simulink model "Finalannfaultdetecandclass"  (R2024b)
settings: Solver=ode45  StartTime=0.0  StopTime=0.4  FixedStep=1e-6  MaxStep=0.04  RelTol=1e-3  EnableMultiTasking=on
PreLoadFcn:
  | power_13NodeTestFeeder_init;
values from neighbouring files (symbols this model uses):
  C_601 = [1.03835973183e-08  -3.28956213337e-09  -2.07596127216e-09; -3.28956213337e-09  9.8230300863e-09  -1.22250137004e-09; -2.07596127216e-09  -1.22250137004e-09  9.29377945947e-09]    [Finalmat.mat]    (also in bus1.mat; bus10.mat; bus11.mat; bus12.mat)
  C_602 = [9.39333329896e-09  -1.78290377777e-09  -2.78635373607e-09; -1.78290377777e-09  8.5370713848e-09  -1.08586207709e-09; -2.78635373607e-09  -1.08586207709e-09  8.94105559107e-09]    [Finalmat.mat]    (also in bus1.mat; bus10.mat; bus11.mat; bus12.mat)
  C_603 = [0  0  0; 0  7.76272711671e-09  -1.48325331387e-09; 0  -1.48325331387e-09  7.69036927641e-09]    [Finalmat.mat]    (also in bus1.mat; bus10.mat; bus11.mat; bus12.mat)
  C_604 = [7.69036927641e-09  0  -1.48325331387e-09; 0  0  0; -1.48325331387e-09  0  7.76272711671e-09]    [Finalmat.mat]    (also in bus1.mat; bus10.mat; bus11.mat; bus12.mat)
  C_605 = [0  0  0; 0  0  0; 0  0  7.44890176838e-09]    [Finalmat.mat]    (also in bus1.mat; bus10.mat; bus11.mat; bus12.mat)
  C_606 = [1.59697709306e-07  -1.64824237567e-15  -1.64824237567e-15; -1.64824237567e-15  1.59697709306e-07  -1.64824237567e-15; -1.64824237567e-15  -1.64824237567e-15  1.59697709306e-07]    [Finalmat.mat]    (also in bus1.mat; bus10.mat; bus11.mat; bus12.mat)
  C_607 = [1.46679066902e-07  0  0; 0  0  0; 0  0  0]    [Finalmat.mat]    (also in bus1.mat; bus10.mat; bus11.mat; bus12.mat)
  ft2km = 0.0003048    [Finalmat.mat]    (also in bus1.mat; bus10.mat; bus11.mat; bus12.mat)
  L_601 = [0.0016777459142  0.000826923199875  0.000698195470335; 0.000826923199875  0.00172702836123  0.000634408490396; 0.000698195470335  0.000634408490396  0.00170560121035]    [Finalmat.mat]    (also in bus1.mat; bus10.mat; bus11.mat; bus12.mat)
  L_602 = [0.00194723354262  0.000698195470335  0.000826923199875; 0.000698195470335  0.00197508883877  0.000634408490396; 0.000826923199875  0.000634408490396  0.00199635116541]    [Finalmat.mat]    (also in bus1.mat; bus10.mat; bus11.mat; bus12.mat)
  L_603 = [0  0  0; 0  0.00222034730427  0.000756708074671; 0  0.000756708074671  0.00223650007955]    [Finalmat.mat]    (also in bus1.mat; bus10.mat; bus11.mat; bus12.mat)
  L_604 = [0.00223650007955  0  0.000756708074671; 0  0  0; 0.000756708074671  0  0.00222034730427]    [Finalmat.mat]    (also in bus1.mat; bus10.mat; bus11.mat; bus12.mat)
  L_605 = [0  0  0; 0  0  0; 0  0  0.00222100660122]    [Finalmat.mat]    (also in bus1.mat; bus10.mat; bus11.mat; bus12.mat)
  L_606 = [0.000735610572263  5.40623499221e-05  2.35698659721e-05; 5.40623499221e-05  0.000666054744009  5.40623499221e-05; 2.35698659721e-05  5.40623499221e-05  0.000735610572263]    [Finalmat.mat]    (also in bus1.mat; bus10.mat; bus11.mat; bus12.mat)
  L_607 = [0.000844559393295  0  0; 0  0  0; 0  0  0]    [Finalmat.mat]    (also in bus1.mat; bus10.mat; bus11.mat; bus12.mat)
  R_601 = [0.215305653249  0.0969341469174  0.0981768923907; 0.0969341469174  0.209713298619  0.0953807150757; 0.0981768923907  0.0953807150757  0.212136652292]    [Finalmat.mat]    (also in bus1.mat; bus10.mat; bus11.mat; bus12.mat)
  R_602 = [0.467645121603  0.0981768923907  0.0969341469174; 0.0981768923907  0.464476120646  0.0953807150757; 0.0969341469174  0.0953807150757  0.462052766973]    [Finalmat.mat]    (also in bus1.mat; bus10.mat; bus11.mat; bus12.mat)
  R_603 = [0  0  0; 0  0.826052916102  0.128375607392; 0  0.128375607392  0.822573228777]    [Finalmat.mat]    (also in bus1.mat; bus10.mat; bus11.mat; bus12.mat)
  R_604 = [0.822573228777  0  0.128375607392; 0  0  0; 0.128375607392  0  0.826052916102]    [Finalmat.mat]    (also in bus1.mat; bus10.mat; bus11.mat; bus12.mat)
  R_605 = [0  0  0; 0  0  0; 0  0  0.825928641555]    [Finalmat.mat]    (also in bus1.mat; bus10.mat; bus11.mat; bus12.mat)
  R_606 = [0.495979718394  0.198342177539  0.177029092672; 0.198342177539  0.49032522649  0.198342177539; 0.177029092672  0.198342177539  0.495979718394]    [Finalmat.mat]    (also in bus1.mat; bus10.mat; bus11.mat; bus12.mat)
  R_607 = [0.834192898952  0  0; 0  0  0; 0  0  0]    [Finalmat.mat]    (also in bus1.mat; bus10.mat; bus11.mat; bus12.mat)
libraries: neural x123, spsLoadFlowBusLib x12, spsDistributedParametersLineLib x9, spsThreePhaseSeriesRLCLoadLib x7, spsMultimeterLib x6, spsPowerPhasorLib x6, spsSeriesRLCLoadLib x5, spsThreePhaseVIMeasurementLib x4, spsGroundLib x4, spsThreePhaseSourceLib x1, spsThreePhaseBreakerLib x1, simulink x1
(part 3 of 4)

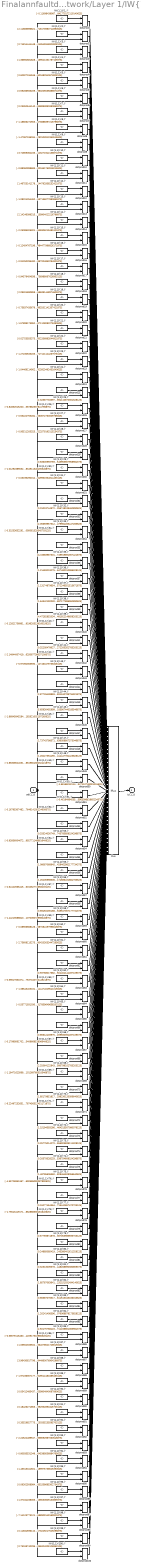
== system Finalannfaultdetecandclass/Subsystem1/Function Fitting Neural Network/Layer 1/IW{1,1} ==
  "pd{1,1}" : Inport  PortDimensions=9
      mask Display: e = 0.06;c1 = [120 230 180]/255;c2 = ([120 230 180]+0)/(256+128);c3 = ([120 230 180]+128)/(256+128);patch([0 1 1 0],[0 0 1 1],c1);patch([0 1 1 1-e 1-e 0+e],[0 0 1 1-e 0+e 0+e],c2);patch([0 0 1 1-e 0+e 0+e],[0 1 1 1-e 1-e 0+e],c3);plot([0 1 1 0 0],[0 0 1 1 0]);
  "IW{1,1}(1,:)'" : Constant  Value=[-0.1169843998710173860189343031379394233226776123046875;-0.315271633824277086599607855532667599618434906005859375;0.79107230882120094239695617943652905523777008056640625;2.164746661655950532576753175817430019378662109375;2.22846879307639600398260881775058805942535400390625;-0.496204760157834379175056938038324005901813507080078125;0.789299834193724958453231010935269296169281005859375;1.6089462914118823899656263165525160729885101318359375;1.6317914608558441447172526750364340841770172119140625]
      mask Display: e = 0.06;c1 = [120 150 230]/255;c2 = ([120 150 230]+0)/383;c3 = ([120 150 230]+128)/383;patch([0 1 1 0],[0 0 1 1],c1);patch([0 1 1 1-e 1-e 0+e],[0 0 1 1-e 0+e 0+e],c2);patch([0 0 1 1-e 0+e 0+e],[0 1 1 1-e 1-e 0+e],c3);plot([0 1 1 0 0],[0 0 1 1 0]);disp('Weights');
  "IW{1,1}(10,:)'" : Constant  Value=[3.7285906223340621323814048082567751407623291015625;-5.223607369509156939102467731572687625885009765625;-3.877261867529044447877595302998088300228118896484375;-2.37152119563655094935938905109651386737823486328125;0.346269172224675625404444190280628390610218048095703125;0.249853727006402959176512013073079288005828857421875;2.016518874910780301235035949503071606159210205078125;0.12714323667959070984778691126848571002483367919921875;3.85153838870149467510373142431490123271942138671875]
      mask Display: e = 0.06;c1 = [120 150 230]/255;c2 = ([120 150 230]+0)/383;c3 = ([120 150 230]+128)/383;patch([0 1 1 0],[0 0 1 1],c1);patch([0 1 1 1-e 1-e 0+e],[0 0 1 1-e 0+e 0+e],c2);patch([0 0 1 1-e 0+e 0+e],[0 1 1 1-e 1-e 0+e],c3);plot([0 1 1 0 0],[0 0 1 1 0]);disp('Weights');
  "IW{1,1}(100,:)'" : Constant  Value=[0.75159740295858845637866352262790314853191375732421875;0.611763010254613437410853293840773403644561767578125;-1.1757815630723575939242664389894343912601470947265625;-0.3695637396224269455302646747441031038761138916015625;-1.00856355672777286969221677281893789768218994140625;-1.17072870773329018589947736472822725772857666015625;-0.284274780055891851393568003913969732820987701416015625;-0.27928563589691524082780915705370716750621795654296875;-0.460633928950748672281889639634755440056324005126953125]
      mask Display: e = 0.06;c1 = [120 150 230]/255;c2 = ([120 150 230]+0)/383;c3 = ([120 150 230]+128)/383;patch([0 1 1 0],[0 0 1 1],c1);patch([0 1 1 1-e 1-e 0+e],[0 0 1 1-e 0+e 0+e],c2);patch([0 0 1 1-e 0+e 0+e],[0 1 1 1-e 1-e 0+e],c3);plot([0 1 1 0 0],[0 0 1 1 0]);disp('Weights');
  "IW{1,1}(11,:)'" : Constant  Value=[-0.8806299868369491523623082684935070574283599853515625;0.30294503373344217056484239947167225182056427001953125;-0.985643459112008457623232970945537090301513671875;-1.042790592220203205187090134131722152233123779296875;0.03439230691604992784515815174017916433513164520263671875;-0.7663674282703316631426559979445300996303558349609375;-0.1309829792505974033200999429027433507144451141357421875;1.19695760712173449036299643921665847301483154296875;-0.603326884093489557159273317665793001651763916015625]
      mask Display: e = 0.06;c1 = [120 150 230]/255;c2 = ([120 150 230]+0)/383;c3 = ([120 150 230]+128)/383;patch([0 1 1 0],[0 0 1 1],c1);patch([0 1 1 1-e 1-e 0+e],[0 0 1 1-e 0+e 0+e],c2);patch([0 0 1 1-e 0+e 0+e],[0 1 1 1-e 1-e 0+e],c3);plot([0 1 1 0 0],[0 0 1 1 0]);disp('Weights');
  "IW{1,1}(12,:)'" : Constant  Value=[1.467531411784743777815265275421552360057830810546875;0.81942273041387891918674313274095766246318817138671875;-0.426906460314266433808683132156147621572017669677734375;0.0749099326592369274546712176743312738835811614990234375;0.2767354436636242365210591742652468383312225341796875;-0.44931784033513844089924305080785416066646575927734375;-1.3652143765277269249480696089449338614940643310546875;-0.9067069902855917629125315215787850320339202880859375;1.80456787422012165933438154752366244792938232421875]
      mask Display: e = 0.06;c1 = [120 150 230]/255;c2 = ([120 150 230]+0)/383;c3 = ([120 150 230]+128)/383;patch([0 1 1 0],[0 0 1 1],c1);patch([0 1 1 1-e 1-e 0+e],[0 0 1 1-e 0+e 0+e],c2);patch([0 0 1 1-e 0+e 0+e],[0 1 1 1-e 1-e 0+e],c3);plot([0 1 1 0 0],[0 0 1 1 0]);disp('Weights');
  "IW{1,1}(13,:)'" : Constant  Value=[-1.0822425445261616427927719996660016477108001708984375;0.1421490865617053567238059486044221557676792144775390625;-0.222184322552897717262254673187271691858768463134765625;-0.808228806975540781110112220630981028079986572265625;-1.0680830130463825344833139752154238522052764892578125;-0.601523564092997897745362934074364602565765380859375;-0.383432119718707775657406955360784195363521575927734375;-0.9219141055654793692752946299151517450809478759765625;0.8695716425988064823826562133035622537136077880859375]
      mask Display: e = 0.06;c1 = [120 150 230]/255;c2 = ([120 150 230]+0)/383;c3 = ([120 150 230]+128)/383;patch([0 1 1 0],[0 0 1 1],c1);patch([0 1 1 1-e 1-e 0+e],[0 0 1 1-e 0+e 0+e],c2);patch([0 0 1 1-e 0+e 0+e],[0 1 1 1-e 1-e 0+e],c3);plot([0 1 1 0 0],[0 0 1 1 0]);disp('Weights');
  "IW{1,1}(14,:)'" : Constant  Value=[2.142460993155533177656479892903007566928863525390625;10.1614423157743711811917819431982934474945068359375;3.70307782718048716930070440866984426975250244140625;-3.40332227325013025875932726194150745868682861328125;-4.92901742923601204893202520906925201416015625;-0.3106434304567471382796384204993955790996551513671875;0.36314955798367598571729786272044293582439422607421875;-1.5022598816808301336322983843274414539337158203125;-0.85323991640809271341794328691321425139904022216796875]
      mask Display: e = 0.06;c1 = [120 150 230]/255;c2 = ([120 150 230]+0)/383;c3 = ([120 150 230]+128)/383;patch([0 1 1 0],[0 0 1 1],c1);patch([0 1 1 1-e 1-e 0+e],[0 0 1 1-e 0+e 0+e],c2);patch([0 0 1 1-e 0+e 0+e],[0 1 1 1-e 1-e 0+e],c3);plot([0 1 1 0 0],[0 0 1 1 0]);disp('Weights');
  "IW{1,1}(15,:)'" : Constant  Value=[-2.250853263014513050421783191268332302570343017578125;-1.5675733809487208958444171003066003322601318359375;-2.639720797748891012446392778656445443630218505859375;-1.129364156634995453032388468272984027862548828125;-0.1049300748916680847688809308237978257238864898681640625;-0.46033186696821670746970767140737734735012054443359375;-0.52897352207262049450520180471357889473438262939453125;-0.6865105178810761987762134594959206879138946533203125;-0.829512207131862577824676918680779635906219482421875]
      mask Display: e = 0.06;c1 = [120 150 230]/255;c2 = ([120 150 230]+0)/383;c3 = ([120 150 230]+128)/383;patch([0 1 1 0],[0 0 1 1],c1);patch([0 1 1 1-e 1-e 0+e],[0 0 1 1-e 0+e 0+e],c2);patch([0 0 1 1-e 0+e 0+e],[0 1 1 1-e 1-e 0+e],c3);plot([0 1 1 0 0],[0 0 1 1 0]);disp('Weights');
  "IW{1,1}(16,:)'" : Constant  Value=[-0.124547671966561968037723318047937937080860137939453125;-0.97962320291865012666931988860596902668476104736328125;-0.77587019687066904882755125072435475885868072509765625;-0.79405829690015672372993549288366921246051788330078125;0.908115781658020981836898499750532209873199462890625;-1.15023286167464533491511247120797634124755859375;-0.72788619861410641664889453750220127403736114501953125;-0.6258857474855545888203778304159641265869140625;-0.86503298797361949379336465426604263484477996826171875]
      mask Display: e = 0.06;c1 = [120 150 230]/255;c2 = ([120 150 230]+0)/383;c3 = ([120 150 230]+128)/383;patch([0 1 1 0],[0 0 1 1],c1);patch([0 1 1 1-e 1-e 0+e],[0 0 1 1-e 0+e 0+e],c2);patch([0 0 1 1-e 0+e 0+e],[0 1 1 1-e 1-e 0+e],c3);plot([0 1 1 0 0],[0 0 1 1 0]);disp('Weights');
  "IW{1,1}(17,:)'" : Constant  Value=[-0.9125029549285799124191953524132259190082550048828125;0.65789174760089685900510403371299616992473602294921875;-0.3630280915494610294302901820628903806209564208984375;-1.5262397482698377704224412809708155691623687744140625;0.382282968203021045194844873549300245940685272216796875;-0.50109375420562629610543581293313764035701751708984375;0.403398421119719186034302538246265612542629241943359375;-1.0463958350801878527391863826778717339038848876953125;0.13938267986139585286053943491424433887004852294921875]
      mask Display: e = 0.06;c1 = [120 150 230]/255;c2 = ([120 150 230]+0)/383;c3 = ([120 150 230]+128)/383;patch([0 1 1 0],[0 0 1 1],c1);patch([0 1 1 1-e 1-e 0+e],[0 0 1 1-e 0+e 0+e],c2);patch([0 0 1 1-e 0+e 0+e],[0 1 1 1-e 1-e 0+e],c3);plot([0 1 1 0 0],[0 0 1 1 0]);disp('Weights');
  "IW{1,1}(18,:)'" : Constant  Value=[-0.94579454836057330613385829565231688320636749267578125;-0.481903233177059575620404530127416364848613739013671875;-1.294686789832062867589002053136937320232391357421875;-1.1112375364712818726076193343033082783222198486328125;0.4852736235741639259089197366847656667232513427734375;-0.31209665885055015710491943536908365786075592041015625;-0.475487892830769587337869097609655000269412994384765625;-0.76513410578662643946046273413230665028095245361328125;0.6284181733856375462465848613646812736988067626953125]
      mask Display: e = 0.06;c1 = [120 150 230]/255;c2 = ([120 150 230]+0)/383;c3 = ([120 150 230]+128)/383;patch([0 1 1 0],[0 0 1 1],c1);patch([0 1 1 1-e 1-e 0+e],[0 0 1 1-e 0+e 0+e],c2);patch([0 0 1 1-e 0+e 0+e],[0 1 1 1-e 1-e 0+e],c3);plot([0 1 1 0 0],[0 0 1 1 0]);disp('Weights');
  "IW{1,1}(19,:)'" : Constant  Value=[2.09324690859917073026963407755829393863677978515625;1.8545893594789186753502008286886848509311676025390625;3.40226567513793387576015447848476469516754150390625;1.990023753797214300931273101014085114002227783203125;3.124260085397577046961714586359448730945587158203125;3.325679193829385926761688097030855715274810791015625;2.143373231000686107705632821307517588138580322265625;4.98029780353131013015399730647914111614227294921875;-0.0279620074952092421971538982461424893699586391448974609375]
      mask Display: e = 0.06;c1 = [120 150 230]/255;c2 = ([120 150 230]+0)/383;c3 = ([120 150 230]+128)/383;patch([0 1 1 0],[0 0 1 1],c1);patch([0 1 1 1-e 1-e 0+e],[0 0 1 1-e 0+e 0+e],c2);patch([0 0 1 1-e 0+e 0+e],[0 1 1 1-e 1-e 0+e],c3);plot([0 1 1 0 0],[0 0 1 1 0]);disp('Weights');
  "IW{1,1}(2,:)'" : Constant  Value=[2.118838968214732165762370641459710896015167236328125;1.8422898698446019682961605212767608463764190673828125;1.7253980455788096026736866406281478703022003173828125;2.312711415512553880802215644507668912410736083984375;1.633846170213174797680721894721500575542449951171875;3.367708596197346526679439193685539066791534423828125;-0.477140207343875910606101342636975459754467010498046875;2.613116127417966172430396909476257860660552978515625;2.66044281460288178919881829642690718173980712890625]
      mask Display: e = 0.06;c1 = [120 150 230]/255;c2 = ([120 150 230]+0)/383;c3 = ([120 150 230]+128)/383;patch([0 1 1 0],[0 0 1 1],c1);patch([0 1 1 1-e 1-e 0+e],[0 0 1 1-e 0+e 0+e],c2);patch([0 0 1 1-e 0+e 0+e],[0 1 1 1-e 1-e 0+e],c3);plot([0 1 1 0 0],[0 0 1 1 0]);disp('Weights');
  "IW{1,1}(20,:)'" : Constant  Value=[-0.75837435679497067209098304374492727220058441162109375;-0.6892949176616320894339651204063557088375091552734375;0.753111799274041260332523961551487445831298828125;-0.91091131319990059633795453919447027146816253662109375;-1.5778653536172468907494703671545721590518951416015625;0.196715916355157671713271838598302565515041351318359375;-0.741954547816795706438597335363738238811492919921875;-0.72451613103801992821217936580069363117218017578125;0.1524088000274099463648980190555448643863201141357421875]
      mask Display: e = 0.06;c1 = [120 150 230]/255;c2 = ([120 150 230]+0)/383;c3 = ([120 150 230]+128)/383;patch([0 1 1 0],[0 0 1 1],c1);patch([0 1 1 1-e 1-e 0+e],[0 0 1 1-e 0+e 0+e],c2);patch([0 0 1 1-e 0+e 0+e],[0 1 1 1-e 1-e 0+e],c3);plot([0 1 1 0 0],[0 0 1 1 0]);disp('Weights');
  "IW{1,1}(21,:)'" : Constant  Value=[-1.5789917395288621815296892236801795661449432373046875;1.214552039187205334513919297023676335811614990234375;3.73117140937676605716433186898939311504364013671875;0.77037511306426853519013775439816527068614959716796875;1.5764585080023330032616968310321681201457977294921875;2.01224664776738659810462195309810340404510498046875;2.796831728956418405829253970296122133731842041015625;1.3456250197286101499827282168553210794925689697265625;-1.00351996366601614596447689109481871128082275390625]
      mask Display: e = 0.06;c1 = [120 150 230]/255;c2 = ([120 150 230]+0)/383;c3 = ([120 150 230]+128)/383;patch([0 1 1 0],[0 0 1 1],c1);patch([0 1 1 1-e 1-e 0+e],[0 0 1 1-e 0+e 0+e],c2);patch([0 0 1 1-e 0+e 0+e],[0 1 1 1-e 1-e 0+e],c3);plot([0 1 1 0 0],[0 0 1 1 0]);disp('Weights');
  "IW{1,1}(22,:)'" : Constant  Value=[0.0275355537349462921314913188552964129485189914703369140625;1.226104677340150050923739399877376854419708251953125;1.3106202217751985461546837541391141712665557861328125;1.232110528501700219550230031018145382404327392578125;-0.31173567352762432403068260100553743541240692138671875;0.09857858649987212562582072905570385046303272247314453125;0.329183085854514778656465523454244248569011688232421875;-0.5875847517893213467488067180966027081012725830078125;-0.6811877548597073950276126197422854602336883544921875]
      mask Display: e = 0.06;c1 = [120 150 230]/255;c2 = ([120 150 230]+0)/383;c3 = ([120 150 230]+128)/383;patch([0 1 1 0],[0 0 1 1],c1);patch([0 1 1 1-e 1-e 0+e],[0 0 1 1-e 0+e 0+e],c2);patch([0 0 1 1-e 0+e 0+e],[0 1 1 1-e 1-e 0+e],c3);plot([0 1 1 0 0],[0 0 1 1 0]);disp('Weights');
  "IW{1,1}(23,:)'" : Constant  Value=[-1.27230533205212470448941530776210129261016845703125;-0.11966745683074198058903903074678964912891387939453125;0.63457897524731909921769101856625638902187347412109375;-1.3489896876626819022249037516303360462188720703125;0.4505565787059844229389682368491776287555694580078125;-0.97789084951873472828509648024919442832469940185546875;-0.371652066968599259499939080342301167547702789306640625;-1.281336300752595303009684357675723731517791748046875;-1.2393888192458526464889700946514494717121124267578125]
      mask Display: e = 0.06;c1 = [120 150 230]/255;c2 = ([120 150 230]+0)/383;c3 = ([120 150 230]+128)/383;patch([0 1 1 0],[0 0 1 1],c1);patch([0 1 1 1-e 1-e 0+e],[0 0 1 1-e 0+e 0+e],c2);patch([0 0 1 1-e 0+e 0+e],[0 1 1 1-e 1-e 0+e],c3);plot([0 1 1 0 0],[0 0 1 1 0]);disp('Weights');
  "IW{1,1}(24,:)'" : Constant  Value=[-1.0446911490235510910906668868847191333770751953125;-0.271704583611200367609939121393836103379726409912109375;1.759903811105738125064590349211357533931732177734375;0.332299179526138299678450493956916034221649169921875;-0.34729266124596069875707371465978212654590606689453125;-1.04762090118411332895220766658894717693328857421875;1.93106383066935283210341367521323263645172119140625;-0.30132445200165147713988744726520963013172149658203125;1.267073431259236659940370373078621923923492431640625]
      mask Display: e = 0.06;c1 = [120 150 230]/255;c2 = ([120 150 230]+0)/383;c3 = ([120 150 230]+128)/383;patch([0 1 1 0],[0 0 1 1],c1);patch([0 1 1 1-e 1-e 0+e],[0 0 1 1-e 0+e 0+e],c2);patch([0 0 1 1-e 0+e 0+e],[0 1 1 1-e 1-e 0+e],c3);plot([0 1 1 0 0],[0 0 1 1 0]);disp('Weights');
  "IW{1,1}(25,:)'" : Constant  Value=[2.3258773339734784002530432189814746379852294921875;3.05772254680351185385234202840365469455718994140625;2.81110017875498474637652179808355867862701416015625;0.474184669947001313783374598642694763839244842529296875;0.07537300879553054944182122198981232941150665283203125;-0.061881985911661267774075412262391182594001293182373046875;-0.11775935775779833303289478863007389008998870849609375;1.230779610415243308096933105844072997570037841796875;0.60442534998214825225915092232753522694110870361328125]
      mask Display: e = 0.06;c1 = [120 150 230]/255;c2 = ([120 150 230]+0)/383;c3 = ([120 150 230]+128)/383;patch([0 1 1 0],[0 0 1 1],c1);patch([0 1 1 1-e 1-e 0+e],[0 0 1 1-e 0+e 0+e],c2);patch([0 0 1 1-e 0+e 0+e],[0 1 1 1-e 1-e 0+e],c3);plot([0 1 1 0 0],[0 0 1 1 0]);disp('Weights');
  "IW{1,1}(26,:)'" : Constant  Value=[-0.8465251520014482888853990516508929431438446044921875;-0.7411275756970281403113176565966568887233734130859375;-0.401933155944238895695974633781588636338710784912109375;-1.721899964010629613397895809612236917018890380859375;1.1771658564200293550783271712134592235088348388671875;0.0235445106777234063055725954427543911151587963104248046875;0.67866638699933024003740911211934871971607208251953125;0.1939525166064939576404668741815839894115924835205078125;-0.73095004883309389054346638658898882567882537841796875]
      mask Display: e = 0.06;c1 = [120 150 230]/255;c2 = ([120 150 230]+0)/383;c3 = ([120 150 230]+128)/383;patch([0 1 1 0],[0 0 1 1],c1);patch([0 1 1 1-e 1-e 0+e],[0 0 1 1-e 0+e 0+e],c2);patch([0 0 1 1-e 0+e 0+e],[0 1 1 1-e 1-e 0+e],c3);plot([0 1 1 0 0],[0 0 1 1 0]);disp('Weights');
  "IW{1,1}(27,:)'" : Constant  Value=[-0.5522275528407953881782077587558887898921966552734375;-2.089805941907607600427354554994963109493255615234375;-0.97385196919102134938128756402875296771526336669921875;0.0694789617250361757339049972870270721614360809326171875;-1.2692571439475823780185237410478293895721435546875;-0.372321324814063603358960108380415476858615875244140625;-0.379267347674678123592428846677648834884166717529296875;0.402993317242199611261099789771833457052707672119140625;0.00754951907807146528617270320182797149755060672760009765625]
      mask Display: e = 0.06;c1 = [120 150 230]/255;c2 = ([120 150 230]+0)/383;c3 = ([120 150 230]+128)/383;patch([0 1 1 0],[0 0 1 1],c1);patch([0 1 1 1-e 1-e 0+e],[0 0 1 1-e 0+e 0+e],c2);patch([0 0 1 1-e 0+e 0+e],[0 1 1 1-e 1-e 0+e],c3);plot([0 1 1 0 0],[0 0 1 1 0]);disp('Weights');
  "IW{1,1}(28,:)'" : Constant  Value=[-0.9551120532535917195815500235767103731632232666015625;-0.87790956627006921930700400480418466031551361083984375;-1.2151025347190917980100266504450701177120208740234375;-0.93177850512927651305261633751797489821910858154296875;0.43757253186025935054459523598779924213886260986328125;0.9465160594302719498926990127074532210826873779296875;-0.212592857165062987245818248993600718677043914794921875;-0.216523371525882690757924819990876130759716033935546875;-0.56824360668253726114329538177116774022579193115234375]
      mask Display: e = 0.06;c1 = [120 150 230]/255;c2 = ([120 150 230]+0)/383;c3 = ([120 150 230]+128)/383;patch([0 1 1 0],[0 0 1 1],c1);patch([0 1 1 1-e 1-e 0+e],[0 0 1 1-e 0+e 0+e],c2);patch([0 0 1 1-e 0+e 0+e],[0 1 1 1-e 1-e 0+e],c3);plot([0 1 1 0 0],[0 0 1 1 0]);disp('Weights');
  "IW{1,1}(29,:)'" : Constant  Value=[0.6360099375922672049199491084436886012554168701171875;1.4583205073260596673634381659212522208690643310546875;1.066962020950944722841313705430366098880767822265625;-1.0051077032542166111994674793095327913761138916015625;0.378104578422379156155130885963444598019123077392578125;0.5202551325363102829868466869811527431011199951171875;0.391483076205180413609241441008634865283966064453125;1.3262977714431303244424498188891448080539703369140625;0.18827889896320415541453030527918599545955657958984375]
      mask Display: e = 0.06;c1 = [120 150 230]/255;c2 = ([120 150 230]+0)/383;c3 = ([120 150 230]+128)/383;patch([0 1 1 0],[0 0 1 1],c1);patch([0 1 1 1-e 1-e 0+e],[0 0 1 1-e 0+e 0+e],c2);patch([0 0 1 1-e 0+e 0+e],[0 1 1 1-e 1-e 0+e],c3);plot([0 1 1 0 0],[0 0 1 1 0]);disp('Weights');
  "IW{1,1}(3,:)'" : Constant  Value=[0.7481444444870763987864847877062857151031494140625;0.85804440066301845835283756969147361814975738525390625;0.24902555631402656377559878819738514721393585205078125;0.244478470325147079211802747522597201168537139892578125;-0.05035455576940485455939011671944172121584415435791015625;-1.0202597956390508926460825023241341114044189453125;-1.1728054573819524097899602566030807793140411376953125;1.09027501260919645886815487756393849849700927734375;0.99548940560036769387153299248893745243549346923828125]
      mask Display: e = 0.06;c1 = [120 150 230]/255;c2 = ([120 150 230]+0)/383;c3 = ([120 150 230]+128)/383;patch([0 1 1 0],[0 0 1 1],c1);patch([0 1 1 1-e 1-e 0+e],[0 0 1 1-e 0+e 0+e],c2);patch([0 0 1 1-e 0+e 0+e],[0 1 1 1-e 1-e 0+e],c3);plot([0 1 1 0 0],[0 0 1 1 0]);disp('Weights');
  "IW{1,1}(30,:)'" : Constant  Value=[-1.012923890326939524442195761366747319698333740234375;1.03384156601108490036722287186421453952789306640625;0.9660288761139714797110400468227453529834747314453125;0.272303867858178894056919716604170389473438262939453125;-0.27735432713567131912668628501705825328826904296875;0.9281283188652220683678706336650066077709197998046875;0.87804522240845928049424173877923749387264251708984375;0.7492890326621906016413277029641903936862945556640625;0.23566216620405622261813505247118882834911346435546875]
      mask Display: e = 0.06;c1 = [120 150 230]/255;c2 = ([120 150 230]+0)/383;c3 = ([120 150 230]+128)/383;patch([0 1 1 0],[0 0 1 1],c1);patch([0 1 1 1-e 1-e 0+e],[0 0 1 1-e 0+e 0+e],c2);patch([0 0 1 1-e 0+e 0+e],[0 1 1 1-e 1-e 0+e],c3);plot([0 1 1 0 0],[0 0 1 1 0]);disp('Weights');
  "IW{1,1}(31,:)'" : Constant  Value=[-0.03195290012953606872958545181973022408783435821533203125;0.80519448731482923253821581965894438326358795166015625;1.4922090003232717503323101482237689197063446044921875;1.4533859362663010816874020747491158545017242431640625;0.85844917152708166696584157762117683887481689453125;-0.408150383600276056572653260445804335176944732666015625;-0.503014329408599802917478882591240108013153076171875;1.035455398586085262735423384583555161952972412109375;-0.3083181434720974056773457050439901649951934814453125]
      mask Display: e = 0.06;c1 = [120 150 230]/255;c2 = ([120 150 230]+0)/383;c3 = ([120 150 230]+128)/383;patch([0 1 1 0],[0 0 1 1],c1);patch([0 1 1 1-e 1-e 0+e],[0 0 1 1-e 0+e 0+e],c2);patch([0 0 1 1-e 0+e 0+e],[0 1 1 1-e 1-e 0+e],c3);plot([0 1 1 0 0],[0 0 1 1 0]);disp('Weights');
  "IW{1,1}(32,:)'" : Constant  Value=[0.01019744972784330204473857151015181443654000759124755859375;-0.43434591101068409368934908343362621963024139404296875;-0.025614139650725065155967286045779474079608917236328125;0.8578035772214758214460061935824342072010040283203125;-0.6007658336836076973241915766266174614429473876953125;0.54483529511771233710959450036170892417430877685546875;-1.6888483654419361723597603486268781125545501708984375;-2.107116686179150377711266628466546535491943359375;0.10090901487781202272575598044568323530256748199462890625]
      mask Display: e = 0.06;c1 = [120 150 230]/255;c2 = ([120 150 230]+0)/383;c3 = ([120 150 230]+128)/383;patch([0 1 1 0],[0 0 1 1],c1);patch([0 1 1 1-e 1-e 0+e],[0 0 1 1-e 0+e 0+e],c2);patch([0 0 1 1-e 0+e 0+e],[0 1 1 1-e 1-e 0+e],c3);plot([0 1 1 0 0],[0 0 1 1 0]);disp('Weights');
  "IW{1,1}(33,:)'" : Constant  Value=[2.056599575128888801600623992271721363067626953125;2.110697793572933189665263853385113179683685302734375;1.9109298626065107651328389692935161292552947998046875;1.37841441391478980449392111040651798248291015625;0.963341731064137007933823042549192905426025390625;0.48665610488103883124466619847225956618785858154296875;1.522029097578674328161696394090540707111358642578125;2.11443286762879978368800948373973369598388671875;0.2442990813332394373080802552067325450479984283447265625]
      mask Display: e = 0.06;c1 = [120 150 230]/255;c2 = ([120 150 230]+0)/383;c3 = ([120 150 230]+128)/383;patch([0 1 1 0],[0 0 1 1],c1);patch([0 1 1 1-e 1-e 0+e],[0 0 1 1-e 0+e 0+e],c2);patch([0 0 1 1-e 0+e 0+e],[0 1 1 1-e 1-e 0+e],c3);plot([0 1 1 0 0],[0 0 1 1 0]);disp('Weights');
  "IW{1,1}(34,:)'" : Constant  Value=[-0.315336522918347406108097175092552788555622100830078125;-15.8390256035940648615678583155386149883270263671875;-4.28508881048104495192774265888147056102752685546875;1.03338556865256947503439732827246189117431640625;0.862588132970358412165978734265081584453582763671875;1.2985393474270889857535848932457156479358673095703125;10.1934541491762420406530509353615343570709228515625;3.045881240257342970068066279054619371891021728515625;4.638291183885105084527822327800095081329345703125]
      mask Display: e = 0.06;c1 = [120 150 230]/255;c2 = ([120 150 230]+0)/383;c3 = ([120 150 230]+128)/383;patch([0 1 1 0],[0 0 1 1],c1);patch([0 1 1 1-e 1-e 0+e],[0 0 1 1-e 0+e 0+e],c2);patch([0 0 1 1-e 0+e 0+e],[0 1 1 1-e 1-e 0+e],c3);plot([0 1 1 0 0],[0 0 1 1 0]);disp('Weights');
  "IW{1,1}(35,:)'" : Constant  Value=[12.8383987301765021271648947731591761112213134765625;22.477297957753382462442459654994308948516845703125;0.39907143180422621764336099658976309001445770263671875;-3.2035022613544210656755240052007138729095458984375;-4.7037612774220409761483097099699079990386962890625;-1.322687464878381735644552463782019913196563720703125;-14.2999228790693404533840293879620730876922607421875;-1.9095712930794308537230108413496054708957672119140625;-7.80741168209004854361410252749919891357421875]
      mask Display: e = 0.06;c1 = [120 150 230]/255;c2 = ([120 150 230]+0)/383;c3 = ([120 150 230]+128)/383;patch([0 1 1 0],[0 0 1 1],c1);patch([0 1 1 1-e 1-e 0+e],[0 0 1 1-e 0+e 0+e],c2);patch([0 0 1 1-e 0+e 0+e],[0 1 1 1-e 1-e 0+e],c3);plot([0 1 1 0 0],[0 0 1 1 0]);disp('Weights');
  "IW{1,1}(36,:)'" : Constant  Value=[1.2145921927556029285000249728909693658351898193359375;1.1126457804778289162328519523725844919681549072265625;-1.007827229868012874902660769294016063213348388671875;-0.1932226957363692709801483715637004934251308441162109375;-0.73182365372302549122451864604954607784748077392578125;-1.73972472862390414860556120402179658412933349609375;-0.80119066874115330012529057057690806686878204345703125;-0.062241227691445348557675032452607410959899425506591796875;-3.370270234757697824790056984056718647480010986328125]
      mask Display: e = 0.06;c1 = [120 150 230]/255;c2 = ([120 150 230]+0)/383;c3 = ([120 150 230]+128)/383;patch([0 1 1 0],[0 0 1 1],c1);patch([0 1 1 1-e 1-e 0+e],[0 0 1 1-e 0+e 0+e],c2);patch([0 0 1 1-e 0+e 0+e],[0 1 1 1-e 1-e 0+e],c3);plot([0 1 1 0 0],[0 0 1 1 0]);disp('Weights');
  "IW{1,1}(37,:)'" : Constant  Value=[1.131748796549014723922255143406800925731658935546875;-0.4133810753359952183672021419624797999858856201171875;-0.1688921826748999432954434496423345990478992462158203125;0.1597026045481725609054279857446090318262577056884765625;2.24243859723448313303606482804752886295318603515625;2.036455601561022898948749570990912616252899169921875;0.6731409369349943272453629106166772544384002685546875;0.86859697719821638006720831981510855257511138916015625;-0.1574101546435353327080264307369361631572246551513671875]
      mask Display: e = 0.06;c1 = [120 150 230]/255;c2 = ([120 150 230]+0)/383;c3 = ([120 150 230]+128)/383;patch([0 1 1 0],[0 0 1 1],c1);patch([0 1 1 1-e 1-e 0+e],[0 0 1 1-e 0+e 0+e],c2);patch([0 0 1 1-e 0+e 0+e],[0 1 1 1-e 1-e 0+e],c3);plot([0 1 1 0 0],[0 0 1 1 0]);disp('Weights');
  "IW{1,1}(38,:)'" : Constant  Value=[1.6434219203000715037177315025473944842815399169921875;2.226405010047957322427691906341351568698883056640625;1.862115260458557575162785724387504160404205322265625;0.9980324048170980955063669171067886054515838623046875;1.4655459410823248322941481092129833996295928955078125;2.081559498473391389694597819470800459384918212890625;-0.039137346798305085171509887231877655722200870513916015625;0.60295104512200403679145210844581015408039093017578125;5.9311530107843513093257570290006697177886962890625]
      mask Display: e = 0.06;c1 = [120 150 230]/255;c2 = ([120 150 230]+0)/383;c3 = ([120 150 230]+128)/383;patch([0 1 1 0],[0 0 1 1],c1);patch([0 1 1 1-e 1-e 0+e],[0 0 1 1-e 0+e 0+e],c2);patch([0 0 1 1-e 0+e 0+e],[0 1 1 1-e 1-e 0+e],c3);plot([0 1 1 0 0],[0 0 1 1 0]);disp('Weights');
  "IW{1,1}(39,:)'" : Constant  Value=[4.47282852034754085934764589183032512664794921875;14.058330727360118572732972097583115100860595703125;-2.05538484077432226371229262440465390682220458984375;-1.8590883669493589724908133575809188187122344970703125;0.727886994694638023162269746535457670688629150390625;-1.5501939955852630514954171303543262183666229248046875;-10.671813906210292799414673936553299427032470703125;-0.85715509837463244036115384005825035274028778076171875;-2.4006648184319629990568500943481922149658203125]
      mask Display: e = 0.06;c1 = [120 150 230]/255;c2 = ([120 150 230]+0)/383;c3 = ([120 150 230]+128)/383;patch([0 1 1 0],[0 0 1 1],c1);patch([0 1 1 1-e 1-e 0+e],[0 0 1 1-e 0+e 0+e],c2);patch([0 0 1 1-e 0+e 0+e],[0 1 1 1-e 1-e 0+e],c3);plot([0 1 1 0 0],[0 0 1 1 0]);disp('Weights');
  "IW{1,1}(4,:)'" : Constant  Value=[1.36892681828689877221449933131225407123565673828125;0.9188188305955635737376496763317845761775970458984375;-0.1197056617309323611753058003159821964800357818603515625;-1.01477703969053578703096718527376651763916015625;-0.70069608460411103578735492192208766937255859375;0.0386271405669370293534115035072318278253078460693359375;0.450879811862569590541482966727926395833492279052734375;0.72866761663550050354132281427155248820781707763671875;-0.1960104769565419180477050531408167444169521331787109375]
      mask Display: e = 0.06;c1 = [120 150 230]/255;c2 = ([120 150 230]+0)/383;c3 = ([120 150 230]+128)/383;patch([0 1 1 0],[0 0 1 1],c1);patch([0 1 1 1-e 1-e 0+e],[0 0 1 1-e 0+e 0+e],c2);patch([0 0 1 1-e 0+e 0+e],[0 1 1 1-e 1-e 0+e],c3);plot([0 1 1 0 0],[0 0 1 1 0]);disp('Weights');
  "IW{1,1}(40,:)'" : Constant  Value=[-0.1282175686174576167974947793481987901031970977783203125;-1.0073378480415378088963507252628915011882781982421875;-1.2951178312388818003597634742618538439273834228515625;-1.8953323839880595880202918124268762767314910888671875;0.8198626657719516597211395492195151746273040771484375;-1.3124092730480823032479520406923256814479827880859375;0.37353800906434353468199560666107572615146636962890625;-0.5295569001488831251123201582231558859348297119140625;-0.0779617448411723812373708142331452108919620513916015625]
      mask Display: e = 0.06;c1 = [120 150 230]/255;c2 = ([120 150 230]+0)/383;c3 = ([120 150 230]+128)/383;patch([0 1 1 0],[0 0 1 1],c1);patch([0 1 1 1-e 1-e 0+e],[0 0 1 1-e 0+e 0+e],c2);patch([0 0 1 1-e 0+e 0+e],[0 1 1 1-e 1-e 0+e],c3);plot([0 1 1 0 0],[0 0 1 1 0]);disp('Weights');
  "IW{1,1}(41,:)'" : Constant  Value=[0.322054786271240456319020495357108302414417266845703125;1.71551212971519095873418336850591003894805908203125;-1.601917573481291157122541335411369800567626953125;-1.1158403918090316064848366295336745679378509521484375;-2.611198710369861952784731329302303493022918701171875;-2.722712860014073310566118379938416182994842529296875;4.7037228236598007669044818612746894359588623046875;-2.295763476322922880257237920886836946010589599609375;4.6671517962359718723064361256547272205352783203125]
      mask Display: e = 0.06;c1 = [120 150 230]/255;c2 = ([120 150 230]+0)/383;c3 = ([120 150 230]+128)/383;patch([0 1 1 0],[0 0 1 1],c1);patch([0 1 1 1-e 1-e 0+e],[0 0 1 1-e 0+e 0+e],c2);patch([0 0 1 1-e 0+e 0+e],[0 1 1 1-e 1-e 0+e],c3);plot([0 1 1 0 0],[0 0 1 1 0]);disp('Weights');
  "IW{1,1}(42,:)'" : Constant  Value=[-2.148440074195544280399872150155715644359588623046875;-1.0226932692165835447895005927421152591705322265625;0.3885358818840518591031241157907061278820037841796875;0.791303444394999555555614279001019895076751708984375;1.1762517621215600183148808355326764285564422607421875;-1.3515553436655949326450354419648647308349609375;-1.80890751669511473664897494018077850341796875;2.004706291968250564394793400424532592296600341796875;-1.0869402030848041018629146492457948625087738037109375]
      mask Display: e = 0.06;c1 = [120 150 230]/255;c2 = ([120 150 230]+0)/383;c3 = ([120 150 230]+128)/383;patch([0 1 1 0],[0 0 1 1],c1);patch([0 1 1 1-e 1-e 0+e],[0 0 1 1-e 0+e 0+e],c2);patch([0 0 1 1-e 0+e 0+e],[0 1 1 1-e 1-e 0+e],c3);plot([0 1 1 0 0],[0 0 1 1 0]);disp('Weights');
  "IW{1,1}(43,:)'" : Constant  Value=[-5.97092355590941092913226384553126990795135498046875;-4.3346130546679706441182133858092129230499267578125;-1.558963813023808153701565970550291240215301513671875;-3.647627660820671025021511013619601726531982421875;-1.023554174944859784801565183443017303943634033203125;-2.723523889557601052047175471670925617218017578125;-3.28377198915054524519518963643349707126617431640625;-3.408514419542033380139400833286345005035400390625;-1.575560118830367617448473538388498127460479736328125]
      mask Display: e = 0.06;c1 = [120 150 230]/255;c2 = ([120 150 230]+0)/383;c3 = ([120 150 230]+128)/383;patch([0 1 1 0],[0 0 1 1],c1);patch([0 1 1 1-e 1-e 0+e],[0 0 1 1-e 0+e 0+e],c2);patch([0 0 1 1-e 0+e 0+e],[0 1 1 1-e 1-e 0+e],c3);plot([0 1 1 0 0],[0 0 1 1 0]);disp('Weights');
  "IW{1,1}(44,:)'" : Constant  Value=[2.877264388590734522921366078662686049938201904296875;0.58653557382936749586832547720405273139476776123046875;1.908194968820188019975603310740552842617034912109375;-1.3365070935414842256960810118471272289752960205078125;1.0764823585528719984694134836900047957897186279296875;-0.7429934322144402525367468115291558206081390380859375;-0.287583402547373356838988911476917564868927001953125;-0.5447583625360035153306625943514518439769744873046875;0.94924455286198117232032700485433451831340789794921875]
      mask Display: e = 0.06;c1 = [120 150 230]/255;c2 = ([120 150 230]+0)/383;c3 = ([120 150 230]+128)/383;patch([0 1 1 0],[0 0 1 1],c1);patch([0 1 1 1-e 1-e 0+e],[0 0 1 1-e 0+e 0+e],c2);patch([0 0 1 1-e 0+e 0+e],[0 1 1 1-e 1-e 0+e],c3);plot([0 1 1 0 0],[0 0 1 1 0]);disp('Weights');
  "IW{1,1}(45,:)'" : Constant  Value=[5.65930492999350320815210579894483089447021484375;5.16564236145193245164364270749501883983612060546875;6.7424469755673523962968829437159001827239990234375;2.162834107263791327824264953960664570331573486328125;3.9968791077088301477715504006482660770416259765625;2.3997657131036600475226805428974330425262451171875;2.562097160760552494451758320792578160762786865234375;1.7918513519749890150478677242062985897064208984375;0.5847972865935797681657959401491098105907440185546875]
      mask Display: e = 0.06;c1 = [120 150 230]/255;c2 = ([120 150 230]+0)/383;c3 = ([120 150 230]+128)/383;patch([0 1 1 0],[0 0 1 1],c1);patch([0 1 1 1-e 1-e 0+e],[0 0 1 1-e 0+e 0+e],c2);patch([0 0 1 1-e 0+e 0+e],[0 1 1 1-e 1-e 0+e],c3);plot([0 1 1 0 0],[0 0 1 1 0]);disp('Weights');
  "IW{1,1}(46,:)'" : Constant  Value=[-1.8684584528486081200782109590363688766956329345703125;-0.6549297470099035844981472109793685376644134521484375;3.665580643705272034793551938491873443126678466796875;2.23633827445562172187010219204239547252655029296875;0.740264669573014177927916534827090799808502197265625;0.4954477786693403107420863307197578251361846923828125;-2.3352894461111333157532499171793460845947265625;2.83586947051348570170148377656005322933197021484375;-2.0840526143699751315807588980533182621002197265625]
      mask Display: e = 0.06;c1 = [120 150 230]/255;c2 = ([120 150 230]+0)/383;c3 = ([120 150 230]+128)/383;patch([0 1 1 0],[0 0 1 1],c1);patch([0 1 1 1-e 1-e 0+e],[0 0 1 1-e 0+e 0+e],c2);patch([0 0 1 1-e 0+e 0+e],[0 1 1 1-e 1-e 0+e],c3);plot([0 1 1 0 0],[0 0 1 1 0]);disp('Weights');
  "IW{1,1}(47,:)'" : Constant  Value=[1.737437985715235555517210741527378559112548828125;1.1065880777431653658737786827259697020053863525390625;1.724479721680829857888284095679409801959991455078125;-0.2861335172744190469273917187820188701152801513671875;2.32165953102500122184892461518757045269012451171875;1.7354145500349396069594831715221516788005828857421875;-0.81170262953208471845556459811632521450519561767578125;2.236994763589100987388746943906880915164947509765625;-4.13387972972960238138284694286994636058807373046875]
      mask Display: e = 0.06;c1 = [120 150 230]/255;c2 = ([120 150 230]+0)/383;c3 = ([120 150 230]+128)/383;patch([0 1 1 0],[0 0 1 1],c1);patch([0 1 1 1-e 1-e 0+e],[0 0 1 1-e 0+e 0+e],c2);patch([0 0 1 1-e 0+e 0+e],[0 1 1 1-e 1-e 0+e],c3);plot([0 1 1 0 0],[0 0 1 1 0]);disp('Weights');
  "IW{1,1}(48,:)'" : Constant  Value=[1.26227394490937339099900782457552850246429443359375;1.5722930552100000678450442137545906007289886474609375;0.326445906793040363513824786423356272280216217041015625;0.6314066239363220756075634199078194797039031982421875;0.63494253069842920833565358407213352620601654052734375;-0.170260047744522025059410452740848995745182037353515625;0.86151667510569251984264838029048405587673187255859375;1.631969390432782773814324173144996166229248046875;-0.566106573098906995511470086057670414447784423828125]
      mask Display: e = 0.06;c1 = [120 150 230]/255;c2 = ([120 150 230]+0)/383;c3 = ([120 150 230]+128)/383;patch([0 1 1 0],[0 0 1 1],c1);patch([0 1 1 1-e 1-e 0+e],[0 0 1 1-e 0+e 0+e],c2);patch([0 0 1 1-e 0+e 0+e],[0 1 1 1-e 1-e 0+e],c3);plot([0 1 1 0 0],[0 0 1 1 0]);disp('Weights');
  "IW{1,1}(49,:)'" : Constant  Value=[-2.86308524031140887444735199096612632274627685546875;-3.40913423280218008670772178447805345058441162109375;-0.88530340833457155103047853117459453642368316650390625;0.2227008046281555297962739814465749077498912811279296875;2.03469862862700257011283611063845455646514892578125;-0.65987901890036460006427887492463923990726470947265625;7.42259266605118295245802073623053729534149169921875;0.2914194840558359533844168254290707409381866455078125;5.51123937470951386075057598645798861980438232421875]
      mask Display: e = 0.06;c1 = [120 150 230]/255;c2 = ([120 150 230]+0)/383;c3 = ([120 150 230]+128)/383;patch([0 1 1 0],[0 0 1 1],c1);patch([0 1 1 1-e 1-e 0+e],[0 0 1 1-e 0+e 0+e],c2);patch([0 0 1 1-e 0+e 0+e],[0 1 1 1-e 1-e 0+e],c3);plot([0 1 1 0 0],[0 0 1 1 0]);disp('Weights');
  "IW{1,1}(5,:)'" : Constant  Value=[0.6292719494691356718618635568418540060520172119140625;3.16979790093921121041375954519025981426239013671875;2.7031945916338013802260320517234504222869873046875;1.6592097592496575231280075968243181705474853515625;0.31882815091059468759482342647970654070377349853515625;2.2162813880736162985840564942918717861175537109375;0.4871916035219399088163072519819252192974090576171875;2.72283157136989562019380173296667635440826416015625;2.061297618227613259733743689139373600482940673828125]
      mask Display: e = 0.06;c1 = [120 150 230]/255;c2 = ([120 150 230]+0)/383;c3 = ([120 150 230]+128)/383;patch([0 1 1 0],[0 0 1 1],c1);patch([0 1 1 1-e 1-e 0+e],[0 0 1 1-e 0+e 0+e],c2);patch([0 0 1 1-e 0+e 0+e],[0 1 1 1-e 1-e 0+e],c3);plot([0 1 1 0 0],[0 0 1 1 0]);disp('Weights');
  "IW{1,1}(50,:)'" : Constant  Value=[-1.6616601311492800174818285086075775325298309326171875;0.8952044794198010801977716255350969731807708740234375;1.321763020856046022544205698068253695964813232421875;3.487150266735332682088710498646833002567291259765625;-0.5209804628258847269961506754043512046337127685546875;-0.025482221909901396628139735867080162279307842254638671875;-1.1454334185730850048656748185749165713787078857421875;-3.952598369489914720276146908872760832309722900390625;-1.8707694793105018593593058540136553347110748291015625]
      mask Display: e = 0.06;c1 = [120 150 230]/255;c2 = ([120 150 230]+0)/383;c3 = ([120 150 230]+128)/383;patch([0 1 1 0],[0 0 1 1],c1);patch([0 1 1 1-e 1-e 0+e],[0 0 1 1-e 0+e 0+e],c2);patch([0 0 1 1-e 0+e 0+e],[0 1 1 1-e 1-e 0+e],c3);plot([0 1 1 0 0],[0 0 1 1 0]);disp('Weights');
  "IW{1,1}(51,:)'" : Constant  Value=[-0.4618486453548802384005966814584098756313323974609375;-0.99663121710502966532629898210871033370494842529296875;-0.78497955289230614273066066743922419846057891845703125;-1.16554356530624314558508558548055589199066162109375;-2.50715838187181017104876445955596864223480224609375;-0.71802635002615822212845841931994073092937469482421875;0.04431508133359397805239865419935085810720920562744140625;-1.517751248382927631297434345469810068607330322265625;-1.6268305510436087413239647503360174596309661865234375]
      mask Display: e = 0.06;c1 = [120 150 230]/255;c2 = ([120 150 230]+0)/383;c3 = ([120 150 230]+128)/383;patch([0 1 1 0],[0 0 1 1],c1);patch([0 1 1 1-e 1-e 0+e],[0 0 1 1-e 0+e 0+e],c2);patch([0 0 1 1-e 0+e 0+e],[0 1 1 1-e 1-e 0+e],c3);plot([0 1 1 0 0],[0 0 1 1 0]);disp('Weights');
  "IW{1,1}(52,:)'" : Constant  Value=[-0.167953074823381232061336731931078247725963592529296875;0.51157971359619403006746551909600384533405303955078125;1.2520227774846397483798909888719208538532257080078125;-0.2318961708506734054058284755228669382631778717041015625;0.0845318422466766750122957319035776890814304351806640625;1.1192568142812084897030899810488335788249969482421875;1.693081525347308602391649401397444307804107666015625;-0.464853614295640815701204928700462915003299713134765625;0.0199039367802343568347733793189036077819764614105224609375]
      mask Display: e = 0.06;c1 = [120 150 230]/255;c2 = ([120 150 230]+0)/383;c3 = ([120 150 230]+128)/383;patch([0 1 1 0],[0 0 1 1],c1);patch([0 1 1 1-e 1-e 0+e],[0 0 1 1-e 0+e 0+e],c2);patch([0 0 1 1-e 0+e 0+e],[0 1 1 1-e 1-e 0+e],c3);plot([0 1 1 0 0],[0 0 1 1 0]);disp('Weights');
  "IW{1,1}(53,:)'" : Constant  Value=[0.3332403074943226517490302285295911133289337158203125;0.10630438559146894450524456487983115948736667633056640625;1.2385015739982689897402678980142809450626373291015625;0.98284621777113911900158882417599670588970184326171875;1.13221220494092822406173581839539110660552978515625;-1.26154527795133564183061025687493383884429931640625;0.1807014850310235676289494222146458923816680908203125;-0.89941880132014662141415328733273781836032867431640625;-0.5017159499482548579152307866024784743785858154296875]
      mask Display: e = 0.06;c1 = [120 150 230]/255;c2 = ([120 150 230]+0)/383;c3 = ([120 150 230]+128)/383;patch([0 1 1 0],[0 0 1 1],c1);patch([0 1 1 1-e 1-e 0+e],[0 0 1 1-e 0+e 0+e],c2);patch([0 0 1 1-e 0+e 0+e],[0 1 1 1-e 1-e 0+e],c3);plot([0 1 1 0 0],[0 0 1 1 0]);disp('Weights');
  "IW{1,1}(54,:)'" : Constant  Value=[-0.93936004672923101299630843641352839767932891845703125;1.540222930941651302561012926162220537662506103515625;0.52905125581045731042451052417163737118244171142578125;0.82376667467047137716207316771033219993114471435546875;0.18390842715059374512520662392489612102508544921875;0.176725442956407630124004981553298421204090118408203125;1.2543611557792557764656748986453749239444732666015625;-0.445294837186404002249417999337310902774333953857421875;-0.3264799659135066978166150875040329992771148681640625]
      mask Display: e = 0.06;c1 = [120 150 230]/255;c2 = ([120 150 230]+0)/383;c3 = ([120 150 230]+128)/383;patch([0 1 1 0],[0 0 1 1],c1);patch([0 1 1 1-e 1-e 0+e],[0 0 1 1-e 0+e 0+e],c2);patch([0 0 1 1-e 0+e 0+e],[0 1 1 1-e 1-e 0+e],c3);plot([0 1 1 0 0],[0 0 1 1 0]);disp('Weights');
  "IW{1,1}(55,:)'" : Constant  Value=[1.0808706894556523447903373380540870130062103271484375;0.11632583299965022771704781234802794642746448516845703125;1.23022439885960199745795762282796204090118408203125;1.545607475311957745844892997411079704761505126953125;-0.312348135661560666331837410325533710420131683349609375;-0.06299657028277737269572611467083333991467952728271484375;0.272784918172833179550451632167096249759197235107421875;-2.407669650771854019666307067382149398326873779296875;-2.9729945222930975745612158789299428462982177734375]
      mask Display: e = 0.06;c1 = [120 150 230]/255;c2 = ([120 150 230]+0)/383;c3 = ([120 150 230]+128)/383;patch([0 1 1 0],[0 0 1 1],c1);patch([0 1 1 1-e 1-e 0+e],[0 0 1 1-e 0+e 0+e],c2);patch([0 0 1 1-e 0+e 0+e],[0 1 1 1-e 1-e 0+e],c3);plot([0 1 1 0 0],[0 0 1 1 0]);disp('Weights');
  "IW{1,1}(56,:)'" : Constant  Value=[1.2520599850645195427745193228474818170070648193359375;-0.1564858341334803004674114390581962652504444122314453125;-0.8773358319586659348487955867312848567962646484375;1.0134751098854730688714198549860157072544097900390625;2.830661200482635475594861418358050286769866943359375;1.7227091493954616030492843492538668215274810791015625;2.3824342960496505128276112372986972332000732421875;1.376967009905302408157012905576266348361968994140625;0.7944206865990131039012567271129228174686431884765625]
      mask Display: e = 0.06;c1 = [120 150 230]/255;c2 = ([120 150 230]+0)/383;c3 = ([120 150 230]+128)/383;patch([0 1 1 0],[0 0 1 1],c1);patch([0 1 1 1-e 1-e 0+e],[0 0 1 1-e 0+e 0+e],c2);patch([0 0 1 1-e 0+e 0+e],[0 1 1 1-e 1-e 0+e],c3);plot([0 1 1 0 0],[0 0 1 1 0]);disp('Weights');
  "IW{1,1}(57,:)'" : Constant  Value=[-2.641225664155180563597014042898081243038177490234375;-0.485357846697780204170413753672619350254535675048828125;0.336540999308858612693029499496333301067352294921875;0.07254716763710467031245343605405651032924652099609375;-1.700349645335781811894548809505067765712738037109375;-0.487460327225782530380371326828026212751865386962890625;-1.8372936484108557397831873458926565945148468017578125;-1.7856661738337129552434134893701411783695220947265625;-1.1393011531118599766188026478630490601062774658203125]
      mask Display: e = 0.06;c1 = [120 150 230]/255;c2 = ([120 150 230]+0)/383;c3 = ([120 150 230]+128)/383;patch([0 1 1 0],[0 0 1 1],c1);patch([0 1 1 1-e 1-e 0+e],[0 0 1 1-e 0+e 0+e],c2);patch([0 0 1 1-e 0+e 0+e],[0 1 1 1-e 1-e 0+e],c3);plot([0 1 1 0 0],[0 0 1 1 0]);disp('Weights');
  "IW{1,1}(58,:)'" : Constant  Value=[0.69450235188456221901986964439856819808483123779296875;-0.20491093813081173724555128501378931105136871337890625;-1.8847453233544990691683551631285808980464935302734375;3.671884101631705643598024835227988660335540771484375;-0.03830043457339012136220190996027668006718158721923828125;3.03139429519694214576475133071653544902801513671875;3.999294034087184090964228744269348680973052978515625;1.8696735426410711067291003928403370082378387451171875;2.514381423842047436068014576449058949947357177734375]
      mask Display: e = 0.06;c1 = [120 150 230]/255;c2 = ([120 150 230]+0)/383;c3 = ([120 150 230]+128)/383;patch([0 1 1 0],[0 0 1 1],c1);patch([0 1 1 1-e 1-e 0+e],[0 0 1 1-e 0+e 0+e],c2);patch([0 0 1 1-e 0+e 0+e],[0 1 1 1-e 1-e 0+e],c3);plot([0 1 1 0 0],[0 0 1 1 0]);disp('Weights');
  "IW{1,1}(59,:)'" : Constant  Value=[-1.442135888407310773118297220207750797271728515625;-1.5867793511257559657678939402103424072265625;1.4355231524617770855201115409727208316326141357421875;-0.85531202860315980185390571932657621800899505615234375;-0.038796938848993323123437448884942568838596343994140625;0.362118298882626865609069000129238702356815338134765625;1.3605001944836008220818257541395723819732666015625;0.12701869272493515605759739628410898149013519287109375;1.6483888183150863238068950522574596107006072998046875]
      mask Display: e = 0.06;c1 = [120 150 230]/255;c2 = ([120 150 230]+0)/383;c3 = ([120 150 230]+128)/383;patch([0 1 1 0],[0 0 1 1],c1);patch([0 1 1 1-e 1-e 0+e],[0 0 1 1-e 0+e 0+e],c2);patch([0 0 1 1-e 0+e 0+e],[0 1 1 1-e 1-e 0+e],c3);plot([0 1 1 0 0],[0 0 1 1 0]);disp('Weights');
  "IW{1,1}(6,:)'" : Constant  Value=[0.5926693320958313915269854987855069339275360107421875;3.0146337754563372612892635515891015529632568359375;-2.788812543508595087615731245023198425769805908203125;0.57404741089781896601351718345540575683116912841796875;-0.64723577508895591137161318329162895679473876953125;0.010087862011053334854171481538287480361759662628173828125;2.87927179499649366078983803163282573223114013671875;-0.1496624801676162130892322466024779714643955230712890625;-1.809507919063463088349408280919305980205535888671875]
      mask Display: e = 0.06;c1 = [120 150 230]/255;c2 = ([120 150 230]+0)/383;c3 = ([120 150 230]+128)/383;patch([0 1 1 0],[0 0 1 1],c1);patch([0 1 1 1-e 1-e 0+e],[0 0 1 1-e 0+e 0+e],c2);patch([0 0 1 1-e 0+e 0+e],[0 1 1 1-e 1-e 0+e],c3);plot([0 1 1 0 0],[0 0 1 1 0]);disp('Weights');
  "IW{1,1}(60,:)'" : Constant  Value=[-0.08906668126857471279311795342437108047306537628173828125;-1.1773770796872806698729618801735341548919677734375;-0.7521855359352020986563047699746675789356231689453125;-1.3726074697805572544240249044378288090229034423828125;-0.487036601578783090449320525294751860201358795166015625;0.401175490536734680180330769871943630278110504150390625;-1.9602966197377396095902213346562348306179046630859375;0.11270097923776851989163816369909909553825855255126953125;-0.10217696571831506868743844052005442790687084197998046875]
      mask Display: e = 0.06;c1 = [120 150 230]/255;c2 = ([120 150 230]+0)/383;c3 = ([120 150 230]+128)/383;patch([0 1 1 0],[0 0 1 1],c1);patch([0 1 1 1-e 1-e 0+e],[0 0 1 1-e 0+e 0+e],c2);patch([0 0 1 1-e 0+e 0+e],[0 1 1 1-e 1-e 0+e],c3);plot([0 1 1 0 0],[0 0 1 1 0]);disp('Weights');
  "IW{1,1}(61,:)'" : Constant  Value=[-2.75608115275438247948613934568129479885101318359375;-2.244394920520104808048245104146189987659454345703125;0.52794249289893058207923104419023729860782623291015625;-0.07703969725674232604806235258365632034838199615478515625;-0.224501778470451107683203417764161713421344757080078125;0.416173564125522699175263596771401353180408477783203125;1.5927708612861073422806157395825721323490142822265625;-0.0097151896662037336149797539519568090327084064483642578125;0.571360772954540241386212073848582804203033447265625]
      mask Display: e = 0.06;c1 = [120 150 230]/255;c2 = ([120 150 230]+0)/383;c3 = ([120 150 230]+128)/383;patch([0 1 1 0],[0 0 1 1],c1);patch([0 1 1 1-e 1-e 0+e],[0 0 1 1-e 0+e 0+e],c2);patch([0 0 1 1-e 0+e 0+e],[0 1 1 1-e 1-e 0+e],c3);plot([0 1 1 0 0],[0 0 1 1 0]);disp('Weights');
  "IW{1,1}(62,:)'" : Constant  Value=[0.93768017682081550301376182687818072736263275146484375;-0.3719233783026678619165750205866061151027679443359375;-0.34521990717194317443983209159341640770435333251953125;0.6764418761884221087399282623664475977420806884765625;-0.71383735835495543131656859259237535297870635986328125;0.451430249976529751609888307939399965107440948486328125;1.51647141394182316531669130199588835239410400390625;1.6310399661724097608583861074293963611125946044921875;0.27774636221241555400496281436062417924404144287109375]
      mask Display: e = 0.06;c1 = [120 150 230]/255;c2 = ([120 150 230]+0)/383;c3 = ([120 150 230]+128)/383;patch([0 1 1 0],[0 0 1 1],c1);patch([0 1 1 1-e 1-e 0+e],[0 0 1 1-e 0+e 0+e],c2);patch([0 0 1 1-e 0+e 0+e],[0 1 1 1-e 1-e 0+e],c3);plot([0 1 1 0 0],[0 0 1 1 0]);disp('Weights');
  "IW{1,1}(63,:)'" : Constant  Value=[-0.5961765167402230947146790640545077621936798095703125;-0.1929164281641480849227576754856272600591182708740234375;-1.567533930999221336577420515823177993297576904296875;0.9830866433600871090447981259785592555999755859375;1.692518089531930503000012322445400059223175048828125;-0.80458574051201947607836473252973519265651702880859375;2.262716109886078630353267726604826748371124267578125;0.43085459696484684766204509287490509450435638427734375;-1.189273527598408985994637987460009753704071044921875]
      mask Display: e = 0.06;c1 = [120 150 230]/255;c2 = ([120 150 230]+0)/383;c3 = ([120 150 230]+128)/383;patch([0 1 1 0],[0 0 1 1],c1);patch([0 1 1 1-e 1-e 0+e],[0 0 1 1-e 0+e 0+e],c2);patch([0 0 1 1-e 0+e 0+e],[0 1 1 1-e 1-e 0+e],c3);plot([0 1 1 0 0],[0 0 1 1 0]);disp('Weights');
  "IW{1,1}(64,:)'" : Constant  Value=[-1.3864340316183259016469264679471962153911590576171875;-2.17042720636273855916442698799073696136474609375;-4.3776116350380380737306040828116238117218017578125;-1.1458568696088773375407754429033957421779632568359375;-1.09314683024334868832738720811903476715087890625;-0.289420486385802699924596481650951318442821502685546875;-5.56816159430000201524535441421903669834136962890625;-0.82404256990567870122532667664927430450916290283203125;-2.7533470909466846165969400317408144474029541015625]
      mask Display: e = 0.06;c1 = [120 150 230]/255;c2 = ([120 150 230]+0)/383;c3 = ([120 150 230]+128)/383;patch([0 1 1 0],[0 0 1 1],c1);patch([0 1 1 1-e 1-e 0+e],[0 0 1 1-e 0+e 0+e],c2);patch([0 0 1 1-e 0+e 0+e],[0 1 1 1-e 1-e 0+e],c3);plot([0 1 1 0 0],[0 0 1 1 0]);disp('Weights');
  "IW{1,1}(65,:)'" : Constant  Value=[-0.55771931030168964138482579073752276599407196044921875;-0.806190441518300104917216231115162372589111328125;-0.99362375143691716861127360971295274794101715087890625;0.28449027835009610409855440593673847615718841552734375;-0.99790166195604024235166207290603779256343841552734375;-0.7482475900580276562124026895617134869098663330078125;-1.0663304649944524982174698379822075366973876953125;0.26786559286164079995984366178163327276706695556640625;-0.83132309939701098944198065510136075317859649658203125]
      mask Display: e = 0.06;c1 = [120 150 230]/255;c2 = ([120 150 230]+0)/383;c3 = ([120 150 230]+128)/383;patch([0 1 1 0],[0 0 1 1],c1);patch([0 1 1 1-e 1-e 0+e],[0 0 1 1-e 0+e 0+e],c2);patch([0 0 1 1-e 0+e 0+e],[0 1 1 1-e 1-e 0+e],c3);plot([0 1 1 0 0],[0 0 1 1 0]);disp('Weights');
  "IW{1,1}(66,:)'" : Constant  Value=[0.856124039754881049901769074494950473308563232421875;-0.67608088075919015036419068565010093152523040771484375;-1.4017620219559694394462212585494853556156158447265625;-0.2551573969081168957728777968441136181354522705078125;-0.68701931566954266283886454402818344533443450927734375;0.309940422571772289384028908898471854627132415771484375;0.327810055841501746254351701281848363578319549560546875;-1.4586004583038121307225765121984295547008514404296875;-0.375602683033563200520887903621769510209560394287109375]
      mask Display: e = 0.06;c1 = [120 150 230]/255;c2 = ([120 150 230]+0)/383;c3 = ([120 150 230]+128)/383;patch([0 1 1 0],[0 0 1 1],c1);patch([0 1 1 1-e 1-e 0+e],[0 0 1 1-e 0+e 0+e],c2);patch([0 0 1 1-e 0+e 0+e],[0 1 1 1-e 1-e 0+e],c3);plot([0 1 1 0 0],[0 0 1 1 0]);disp('Weights');
  "IW{1,1}(67,:)'" : Constant  Value=[-0.1799956170298237234650429172688745893537998199462890625;1.1470541567788925529924881629995070397853851318359375;-0.50366333715227129541602835161029361188411712646484375;0.9155625535363884903716780172544531524181365966796875;-0.9913078603875578043158611762919463217258453369140625;-0.281674444323168515769140185511787422001361846923828125;0.78530933526400958921698247650056146085262298583984375;1.342170933417862865866254651336930692195892333984375;0.64609064385422387832846879973658360540866851806640625]
      mask Display: e = 0.06;c1 = [120 150 230]/255;c2 = ([120 150 230]+0)/383;c3 = ([120 150 230]+128)/383;patch([0 1 1 0],[0 0 1 1],c1);patch([0 1 1 1-e 1-e 0+e],[0 0 1 1-e 0+e 0+e],c2);patch([0 0 1 1-e 0+e 0+e],[0 1 1 1-e 1-e 0+e],c3);plot([0 1 1 0 0],[0 0 1 1 0]);disp('Weights');
  "IW{1,1}(68,:)'" : Constant  Value=[2.320641228437746672597086217137984931468963623046875;5.3733709201662218646333712968043982982635498046875;2.61009972835581383066028138273395597934722900390625;0.30528449408072522164303563840803690254688262939453125;0.68983538011284384339205644209869205951690673828125;1.39684811369063499597586996969766914844512939453125;-1.03220780825192637308873599977232515811920166015625;0.5091892303853968737570312441675923764705657958984375;3.17102312795787799615254698437638580799102783203125]
      mask Display: e = 0.06;c1 = [120 150 230]/255;c2 = ([120 150 230]+0)/383;c3 = ([120 150 230]+128)/383;patch([0 1 1 0],[0 0 1 1],c1);patch([0 1 1 1-e 1-e 0+e],[0 0 1 1-e 0+e 0+e],c2);patch([0 0 1 1-e 0+e 0+e],[0 1 1 1-e 1-e 0+e],c3);plot([0 1 1 0 0],[0 0 1 1 0]);disp('Weights');
  "IW{1,1}(69,:)'" : Constant  Value=[-1.18471623568705819451452043722383677959442138671875;-0.305025993303101816689348879663157276809215545654296875;-0.9353228234794894735415482500684447586536407470703125;-0.12321831376305057703657297452082275412976741790771484375;-1.114721603921468240372405489324592053890228271484375;-1.4666992071371109940258747883490286767482757568359375;-2.40766079614463723856943033752031624317169189453125;2.03055811627409443786973497481085360050201416015625;-1.81269529305818632991531558218412101268768310546875]
      mask Display: e = 0.06;c1 = [120 150 230]/255;c2 = ([120 150 230]+0)/383;c3 = ([120 150 230]+128)/383;patch([0 1 1 0],[0 0 1 1],c1);patch([0 1 1 1-e 1-e 0+e],[0 0 1 1-e 0+e 0+e],c2);patch([0 0 1 1-e 0+e 0+e],[0 1 1 1-e 1-e 0+e],c3);plot([0 1 1 0 0],[0 0 1 1 0]);disp('Weights');
  "IW{1,1}(7,:)'" : Constant  Value=[0.233525441406212841410905411976273171603679656982421875;1.1910777268666137285180184335331432521343231201171875;-0.99601839770604361223860223617521114647388458251953125;0.1056216242047363362832612665442866273224353790283203125;1.234915909367848119160271380678750574588775634765625;0.43462574917993113121639225937542505562305450439453125;-0.81475938165775951826930167953833006322383880615234375;0.79103451236607391638955277812783606350421905517578125;-0.0102818872492788336570068707942482433281838893890380859375]
      mask Display: e = 0.06;c1 = [120 150 230]/255;c2 = ([120 150 230]+0)/383;c3 = ([120 150 230]+128)/383;patch([0 1 1 0],[0 0 1 1],c1);patch([0 1 1 1-e 1-e 0+e],[0 0 1 1-e 0+e 0+e],c2);patch([0 0 1 1-e 0+e 0+e],[0 1 1 1-e 1-e 0+e],c3);plot([0 1 1 0 0],[0 0 1 1 0]);disp('Weights');
  "IW{1,1}(70,:)'" : Constant  Value=[1.8517985181768426006243544179596938192844390869140625;-3.453966940217914949329269802547059953212738037109375;-0.33445863174273327000918243356863968074321746826171875;-1.0467281865373865290536059546866454184055328369140625;1.1826293983087889927219293895177543163299560546875;-1.101726535212721014289627419202588498592376708984375;2.3697880180247476999966238508932292461395263671875;-1.25313335192989949717912168125621974468231201171875;0.72447503133090496163504212745465338230133056640625]
      mask Display: e = 0.06;c1 = [120 150 230]/255;c2 = ([120 150 230]+0)/383;c3 = ([120 150 230]+128)/383;patch([0 1 1 0],[0 0 1 1],c1);patch([0 1 1 1-e 1-e 0+e],[0 0 1 1-e 0+e 0+e],c2);patch([0 0 1 1-e 0+e 0+e],[0 1 1 1-e 1-e 0+e],c3);plot([0 1 1 0 0],[0 0 1 1 0]);disp('Weights');
  "IW{1,1}(71,:)'" : Constant  Value=[-6.224972326510563647161689004860818386077880859375;-4.3587863106178161842763074673712253570556640625;1.8428389968052958369781890723970718681812286376953125;-3.572622835045174749524221624596975743770599365234375;-2.9712723293039591254682818544097244739532470703125;-1.9410926598671995879641372084734030067920684814453125;3.9949554684322858832956626429222524166107177734375;-4.6887848528862772212733034393750131130218505859375;-9.367282026942472583641574601642787456512451171875]
      mask Display: e = 0.06;c1 = [120 150 230]/255;c2 = ([120 150 230]+0)/383;c3 = ([120 150 230]+128)/383;patch([0 1 1 0],[0 0 1 1],c1);patch([0 1 1 1-e 1-e 0+e],[0 0 1 1-e 0+e 0+e],c2);patch([0 0 1 1-e 0+e 0+e],[0 1 1 1-e 1-e 0+e],c3);plot([0 1 1 0 0],[0 0 1 1 0]);disp('Weights');
  "IW{1,1}(72,:)'" : Constant  Value=[1.15194593286558788491902305395342409610748291015625;0.9582685862374347163239463043282739818096160888671875;-0.59297681454480188900646453475928865373134613037109375;-0.07869310063116098652447050199043587781488895416259765625;1.118799429817823209987182053737342357635498046875;1.0446161777566322914623242468223907053470611572265625;-0.419579524670164516475523441840778104960918426513671875;0.53800702339413042363247541288728825747966766357421875;0.56776037013642188799877885685418732464313507080078125]
      mask Display: e = 0.06;c1 = [120 150 230]/255;c2 = ([120 150 230]+0)/383;c3 = ([120 150 230]+128)/383;patch([0 1 1 0],[0 0 1 1],c1);patch([0 1 1 1-e 1-e 0+e],[0 0 1 1-e 0+e 0+e],c2);patch([0 0 1 1-e 0+e 0+e],[0 1 1 1-e 1-e 0+e],c3);plot([0 1 1 0 0],[0 0 1 1 0]);disp('Weights');
  "IW{1,1}(73,:)'" : Constant  Value=[0.257750142703602580507293851042049936950206756591796875;0.292680152494082135294917179635376669466495513916015625;-1.242726850153672568666252118418924510478973388671875;-1.4434984246693780551851205018465407192707061767578125;-0.63532225426459076889074140126467682421207427978515625;-0.41750529958996740464982622142997570335865020751953125;-1.9271737967581514805459619310568086802959442138671875;-0.5571695139522672146625836830935440957546234130859375;-3.89491336629288742443577575613744556903839111328125]
      mask Display: e = 0.06;c1 = [120 150 230]/255;c2 = ([120 150 230]+0)/383;c3 = ([120 150 230]+128)/383;patch([0 1 1 0],[0 0 1 1],c1);patch([0 1 1 1-e 1-e 0+e],[0 0 1 1-e 0+e 0+e],c2);patch([0 0 1 1-e 0+e 0+e],[0 1 1 1-e 1-e 0+e],c3);plot([0 1 1 0 0],[0 0 1 1 0]);disp('Weights');
  "IW{1,1}(74,:)'" : Constant  Value=[0.2057932823393760768393434545942000113427639007568359375;1.228468833083504296865839933161623775959014892578125;1.617851700557862759666249985457397997379302978515625;0.43257976108918894109223174382350407540798187255859375;-0.027870182145089968106521638446793076582252979278564453125;0.667298873639169176641416925122030079364776611328125;0.403807888468451559038641107690636999905109405517578125;3.40767438047778004062138279550708830356597900390625;0.9294704372673894265943772552418522536754608154296875]
      mask Display: e = 0.06;c1 = [120 150 230]/255;c2 = ([120 150 230]+0)/383;c3 = ([120 150 230]+128)/383;patch([0 1 1 0],[0 0 1 1],c1);patch([0 1 1 1-e 1-e 0+e],[0 0 1 1-e 0+e 0+e],c2);patch([0 0 1 1-e 0+e 0+e],[0 1 1 1-e 1-e 0+e],c3);plot([0 1 1 0 0],[0 0 1 1 0]);disp('Weights');
  "IW{1,1}(75,:)'" : Constant  Value=[1.487956063607784873425998739548958837985992431640625;2.610109696397266976219952994142659008502960205078125;0.034383860984059246013178068324123159982264041900634765625;1.208735549149061672125071709160692989826202392578125;0.32591743168935149999043687785160727798938751220703125;-1.280698328166394173166509062866680324077606201171875;-1.452768159872112274655364672071300446987152099609375;1.015246701031779164026147554977796971797943115234375;0.69253886701086886379385987311252392828464508056640625]
      mask Display: e = 0.06;c1 = [120 150 230]/255;c2 = ([120 150 230]+0)/383;c3 = ([120 150 230]+128)/383;patch([0 1 1 0],[0 0 1 1],c1);patch([0 1 1 1-e 1-e 0+e],[0 0 1 1-e 0+e 0+e],c2);patch([0 0 1 1-e 0+e 0+e],[0 1 1 1-e 1-e 0+e],c3);plot([0 1 1 0 0],[0 0 1 1 0]);disp('Weights');
  "IW{1,1}(76,:)'" : Constant  Value=[-4.5572695246769452381840892485342919826507568359375;0.02068756482293833409702443759670131839811801910400390625;-1.688175075094544563825138538959436118602752685546875;-0.40200704820638544223498911378555931150913238525390625;-0.8798287501886665751271721092052757740020751953125;1.0407806972340394313647493618191219866275787353515625;-1.3645216686477763534668383726966567337512969970703125;2.204848914029473139208903376129455864429473876953125;4.29919842654809603033072562539018690586090087890625]
      mask Display: e = 0.06;c1 = [120 150 230]/255;c2 = ([120 150 230]+0)/383;c3 = ([120 150 230]+128)/383;patch([0 1 1 0],[0 0 1 1],c1);patch([0 1 1 1-e 1-e 0+e],[0 0 1 1-e 0+e 0+e],c2);patch([0 0 1 1-e 0+e 0+e],[0 1 1 1-e 1-e 0+e],c3);plot([0 1 1 0 0],[0 0 1 1 0]);disp('Weights');
  "IW{1,1}(77,:)'" : Constant  Value=[0.152774543644878857406865790835581719875335693359375;-0.68679583557578005592603176410193555057048797607421875;1.1249978482455820216756592344609089195728302001953125;0.0381924603162124565169932566277566365897655487060546875;0.7067941007576623579922170392819680273532867431640625;1.1454710832551484589458823393215425312519073486328125;0.3181674525065198988471593111171387135982513427734375;2.7308938785093115342306191450916230678558349609375;-0.627439349640806387498059848439879715442657470703125]
      mask Display: e = 0.06;c1 = [120 150 230]/255;c2 = ([120 150 230]+0)/383;c3 = ([120 150 230]+128)/383;patch([0 1 1 0],[0 0 1 1],c1);patch([0 1 1 1-e 1-e 0+e],[0 0 1 1-e 0+e 0+e],c2);patch([0 0 1 1-e 0+e 0+e],[0 1 1 1-e 1-e 0+e],c3);plot([0 1 1 0 0],[0 0 1 1 0]);disp('Weights');
  "IW{1,1}(78,:)'" : Constant  Value=[-1.7904341917169792619546342393732629716396331787109375;-2.006906523547069554069821606390178203582763671875;-1.2312768544732668463126401547924615442752838134765625;-0.49597588284596183516583778327913023531436920166015625;-0.348600451689187240678080570432939566671848297119140625;-1.1047912770503038881741986187989823520183563232421875;0.684208720358146837980939380940981209278106689453125;-0.411307987556018661567946992363431490957736968994140625;-0.320258733250457228169949530638405121862888336181640625]
      mask Display: e = 0.06;c1 = [120 150 230]/255;c2 = ([120 150 230]+0)/383;c3 = ([120 150 230]+128)/383;patch([0 1 1 0],[0 0 1 1],c1);patch([0 1 1 1-e 1-e 0+e],[0 0 1 1-e 0+e 0+e],c2);patch([0 0 1 1-e 0+e 0+e],[0 1 1 1-e 1-e 0+e],c3);plot([0 1 1 0 0],[0 0 1 1 0]);disp('Weights');
  "IW{1,1}(79,:)'" : Constant  Value=[0.67759874878224024552508808483253233134746551513671875;1.62142526202463699291911325417459011077880859375;2.26606316502667670675918998313136398792266845703125;0.537124924846953621937473144498653709888458251953125;1.6475347335212955357519604149274528026580810546875;0.05829939036981766908862567788673914037644863128662109375;2.37717164455270424383570571080781519412994384765625;0.27318227914492199115414905463694594800472259521484375;0.238688518587205689147623388635111041367053985595703125]
      mask Display: e = 0.06;c1 = [120 150 230]/255;c2 = ([120 150 230]+0)/383;c3 = ([120 150 230]+128)/383;patch([0 1 1 0],[0 0 1 1],c1);patch([0 1 1 1-e 1-e 0+e],[0 0 1 1-e 0+e 0+e],c2);patch([0 0 1 1-e 0+e 0+e],[0 1 1 1-e 1-e 0+e],c3);plot([0 1 1 0 0],[0 0 1 1 0]);disp('Weights');
  "IW{1,1}(8,:)'" : Constant  Value=[-1.188062729039266240960159848327748477458953857421875;-0.92904177396888976137034887869958765804767608642578125;-0.12457332452280191203985992842717678286135196685791015625;0.85047768537227363960795400998904369771480560302734375;-1.0724243677221430015578107486362569034099578857421875;0.477433144902980555190907807627809233963489532470703125;-0.79851786849348460606279331841506063938140869140625;-0.09572787289320584813712144978126161731779575347900390625;-0.479776259563528373330854037703829817473888397216796875]
      mask Display: e = 0.06;c1 = [120 150 230]/255;c2 = ([120 150 230]+0)/383;c3 = ([120 150 230]+128)/383;patch([0 1 1 0],[0 0 1 1],c1);patch([0 1 1 1-e 1-e 0+e],[0 0 1 1-e 0+e 0+e],c2);patch([0 0 1 1-e 0+e 0+e],[0 1 1 1-e 1-e 0+e],c3);plot([0 1 1 0 0],[0 0 1 1 0]);disp('Weights');
  "IW{1,1}(80,:)'" : Constant  Value=[0.248850854197315840554693977537681348621845245361328125;0.624218253690703051006494206376373767852783203125;1.20973935754545269816162544884718954563140869140625;1.39177192685180717290904794936068356037139892578125;0.903224154394205669404982472769916057586669921875;-0.71156567446707075230705186186241917312145233154296875;-0.4585344032652240997549597523175179958343505859375;0.07904699184446713211560364698016201145946979522705078125;0.89036472990428905394111325222183950245380401611328125]
      mask Display: e = 0.06;c1 = [120 150 230]/255;c2 = ([120 150 230]+0)/383;c3 = ([120 150 230]+128)/383;patch([0 1 1 0],[0 0 1 1],c1);patch([0 1 1 1-e 1-e 0+e],[0 0 1 1-e 0+e 0+e],c2);patch([0 0 1 1-e 0+e 0+e],[0 1 1 1-e 1-e 0+e],c3);plot([0 1 1 0 0],[0 0 1 1 0]);disp('Weights');
  "IW{1,1}(81,:)'" : Constant  Value=[0.323130093785219230095862030793796293437480926513671875;-0.4425453026840548975684441757039166986942291259765625;-0.204603533305807883113658363072318024933338165283203125;2.039957712840857251279658157727681100368499755859375;0.58651565071586120314606205283780582249164581298828125;0.67582209467521037193904476225725375115871429443359375;-1.22069787643040950086970042320899665355682373046875;-1.5478009881526071378488040863885544240474700927734375;1.62573156123092843472477397881448268890380859375]
      mask Display: e = 0.06;c1 = [120 150 230]/255;c2 = ([120 150 230]+0)/383;c3 = ([120 150 230]+128)/383;patch([0 1 1 0],[0 0 1 1],c1);patch([0 1 1 1-e 1-e 0+e],[0 0 1 1-e 0+e 0+e],c2);patch([0 0 1 1-e 0+e 0+e],[0 1 1 1-e 1-e 0+e],c3);plot([0 1 1 0 0],[0 0 1 1 0]);disp('Weights');
  "IW{1,1}(82,:)'" : Constant  Value=[1.8578706364157167030271011753939092159271240234375;0.4875865788428839220358668171684257686138153076171875;-0.2091184282980327602263770359058980830013751983642578125;0.47738728004973385310449884855188429355621337890625;0.1730337657418673236175976626327610574662685394287109375;1.867744793148160109552691210410557687282562255859375;0.1716856006757407626661660060563008300960063934326171875;-0.2279918350100330892704647567370557226240634918212890625;1.3718453870996614174515570994117297232151031494140625]
      mask Display: e = 0.06;c1 = [120 150 230]/255;c2 = ([120 150 230]+0)/383;c3 = ([120 150 230]+128)/383;patch([0 1 1 0],[0 0 1 1],c1);patch([0 1 1 1-e 1-e 0+e],[0 0 1 1-e 0+e 0+e],c2);patch([0 0 1 1-e 0+e 0+e],[0 1 1 1-e 1-e 0+e],c3);plot([0 1 1 0 0],[0 0 1 1 0]);disp('Weights');
  "IW{1,1}(83,:)'" : Constant  Value=[0.6558707651799655646840392364538274705410003662109375;0.423406640983424953361691223108209669589996337890625;1.269118907725189870916437939740717411041259765625;-0.7317440363893548127549593118601478636264801025390625;0.181284650598296959156385810274514369666576385498046875;1.203828858975398485853247620980255305767059326171875;0.6858427791366390469107727767550386488437652587890625;1.3512246154535543229968652667594142258167266845703125;0.92254049926797476732787117725820280611515045166015625]
      mask Display: e = 0.06;c1 = [120 150 230]/255;c2 = ([120 150 230]+0)/383;c3 = ([120 150 230]+128)/383;patch([0 1 1 0],[0 0 1 1],c1);patch([0 1 1 1-e 1-e 0+e],[0 0 1 1-e 0+e 0+e],c2);patch([0 0 1 1-e 0+e 0+e],[0 1 1 1-e 1-e 0+e],c3);plot([0 1 1 0 0],[0 0 1 1 0]);disp('Weights');
  "IW{1,1}(84,:)'" : Constant  Value=[1.2024140839684658299546526905032806098461151123046875;0.276102320282240298876530459892819635570049285888671875;0.1309740976456046646081432527353172190487384796142578125;-0.3487879151836164037803200699272565543651580810546875;0.212370705584520980124807465472258627414703369140625;0.086858209890419646459491787027218379080295562744140625;1.42000382642864142468397403717972338199615478515625;1.0236595299815653969943696210975758731365203857421875;0.270328479570696444955757442585309036076068878173828125]
      mask Display: e = 0.06;c1 = [120 150 230]/255;c2 = ([120 150 230]+0)/383;c3 = ([120 150 230]+128)/383;patch([0 1 1 0],[0 0 1 1],c1);patch([0 1 1 1-e 1-e 0+e],[0 0 1 1-e 0+e 0+e],c2);patch([0 0 1 1-e 0+e 0+e],[0 1 1 1-e 1-e 0+e],c3);plot([0 1 1 0 0],[0 0 1 1 0]);disp('Weights');
  "IW{1,1}(85,:)'" : Constant  Value=[2.501757684230345279985385786858387291431427001953125;1.9777596090350739732599549824954010546207427978515625;-0.2419919021076943621562094222099403850734233856201171875;1.987387911766489434484128651092760264873504638671875;2.13055606650560047654607842559926211833953857421875;1.1547764914629576882276751348399557173252105712890625;0.62729997222619837682344723361893557012081146240234375;1.285355689439163118237274829880334436893463134765625;3.35630772895451823245593914180062711238861083984375]
      mask Display: e = 0.06;c1 = [120 150 230]/255;c2 = ([120 150 230]+0)/383;c3 = ([120 150 230]+128)/383;patch([0 1 1 0],[0 0 1 1],c1);patch([0 1 1 1-e 1-e 0+e],[0 0 1 1-e 0+e 0+e],c2);patch([0 0 1 1-e 0+e 0+e],[0 1 1 1-e 1-e 0+e],c3);plot([0 1 1 0 0],[0 0 1 1 0]);disp('Weights');
  "IW{1,1}(86,:)'" : Constant  Value=[-0.585791164605836467416111190686933696269989013671875;-3.18770790502275946920462956768460571765899658203125;-4.9888047173650651444631876074708998203277587890625;1.93910446588226559327949871658347547054290771484375;-1.58258534598469413623433865723200142383575439453125;-0.790598852201497503955351930926553905010223388671875;-0.261434802626678786108271879129461012780666351318359375;1.258124762177846633903754991479218006134033203125;-0.385675725210864073222438719312776811420917510986328125]
      mask Display: e = 0.06;c1 = [120 150 230]/255;c2 = ([120 150 230]+0)/383;c3 = ([120 150 230]+128)/383;patch([0 1 1 0],[0 0 1 1],c1);patch([0 1 1 1-e 1-e 0+e],[0 0 1 1-e 0+e 0+e],c2);patch([0 0 1 1-e 0+e 0+e],[0 1 1 1-e 1-e 0+e],c3);plot([0 1 1 0 0],[0 0 1 1 0]);disp('Weights');
  "IW{1,1}(87,:)'" : Constant  Value=[1.0555233350209720644130584332742728292942047119140625;-0.93242102271713356298477037853444926440715789794921875;-1.1880263551601479843355946286465041339397430419921875;-0.30049278707478166428046506553073413670063018798828125;-0.61398661924565789416163852365571074187755584716796875;0.79417404132231528279817212023772299289703369140625;-0.8247430797428838555873653604066930711269378662109375;0.242078641259022731002659156729350797832012176513671875;0.364411521945056604554480372826219536364078521728515625]
      mask Display: e = 0.06;c1 = [120 150 230]/255;c2 = ([120 150 230]+0)/383;c3 = ([120 150 230]+128)/383;patch([0 1 1 0],[0 0 1 1],c1);patch([0 1 1 1-e 1-e 0+e],[0 0 1 1-e 0+e 0+e],c2);patch([0 0 1 1-e 0+e 0+e],[0 1 1 1-e 1-e 0+e],c3);plot([0 1 1 0 0],[0 0 1 1 0]);disp('Weights');
  "IW{1,1}(88,:)'" : Constant  Value=[3.964308177966085811050334086758084595203399658203125;16.242856030741993578203619108535349369049072265625;3.184608384823464977131379782804287970066070556640625;-0.0305534994510878558926503245629646698944270610809326171875;-0.545315472289350733348101130104623734951019287109375;0.2701762958535105507706930438871495425701141357421875;-15.83441730070641284555676975287497043609619140625;-1.285652235694444645019984818645752966403961181640625;-10.8059310879822003670369667815975844860076904296875]
      mask Display: e = 0.06;c1 = [120 150 230]/255;c2 = ([120 150 230]+0)/383;c3 = ([120 150 230]+128)/383;patch([0 1 1 0],[0 0 1 1],c1);patch([0 1 1 1-e 1-e 0+e],[0 0 1 1-e 0+e 0+e],c2);patch([0 0 1 1-e 0+e 0+e],[0 1 1 1-e 1-e 0+e],c3);plot([0 1 1 0 0],[0 0 1 1 0]);disp('Weights');
  "IW{1,1}(89,:)'" : Constant  Value=[-1.9723635717714265158662101384834386408329010009765625;-0.71187538970598829290992171081597916781902313232421875;1.8122840480279631680815555228036828339099884033203125;1.574850229354618047494795973761938512325286865234375;0.95233906646272092899607741856016218662261962890625;-0.368328750048548647644253151156590320169925689697265625;1.61898394261467526433762031956575810909271240234375;0.497954088565791763709711403862456791102886199951171875;1.841146418085618297055816583451814949512481689453125]
      mask Display: e = 0.06;c1 = [120 150 230]/255;c2 = ([120 150 230]+0)/383;c3 = ([120 150 230]+128)/383;patch([0 1 1 0],[0 0 1 1],c1);patch([0 1 1 1-e 1-e 0+e],[0 0 1 1-e 0+e 0+e],c2);patch([0 0 1 1-e 0+e 0+e],[0 1 1 1-e 1-e 0+e],c3);plot([0 1 1 0 0],[0 0 1 1 0]);disp('Weights');
  "IW{1,1}(9,:)'" : Constant  Value=[-1.470671960348246098959634764469228684902191162109375;-0.37109557269639237286895649958751164376735687255859375;-1.2233280200328715547897218129946850240230560302734375;0.11935766743074606444086072087884531356394290924072265625;-2.239889081462763886776201616157777607440948486328125;-1.6837578239423895976045741917914710938930511474609375;-0.80169345885110476768176113182562403380870819091796875;-0.1393604334602069061421758533469983376562595367431640625;-0.916198494925664963517419892014004290103912353515625]
      mask Display: e = 0.06;c1 = [120 150 230]/255;c2 = ([120 150 230]+0)/383;c3 = ([120 150 230]+128)/383;patch([0 1 1 0],[0 0 1 1],c1);patch([0 1 1 1-e 1-e 0+e],[0 0 1 1-e 0+e 0+e],c2);patch([0 0 1 1-e 0+e 0+e],[0 1 1 1-e 1-e 0+e],c3);plot([0 1 1 0 0],[0 0 1 1 0]);disp('Weights');
  "IW{1,1}(90,:)'" : Constant  Value=[0.05412485437386770070755659389760694466531276702880859375;0.9281079359494908143091151941916905343532562255859375;-0.8875754344005724050248318235389888286590576171875;0.6925177120974501665529032834456302225589752197265625;-0.83880755161971454203495568435755558311939239501953125;0.6596933557169737394332287294673733413219451904296875;-0.06156716612030048441095431144276517443358898162841796875;1.193611121443358680238588931388221681118011474609375;1.1544405209098196340988806696259416639804840087890625]
      mask Display: e = 0.06;c1 = [120 150 230]/255;c2 = ([120 150 230]+0)/383;c3 = ([120 150 230]+128)/383;patch([0 1 1 0],[0 0 1 1],c1);patch([0 1 1 1-e 1-e 0+e],[0 0 1 1-e 0+e 0+e],c2);patch([0 0 1 1-e 0+e 0+e],[0 1 1 1-e 1-e 0+e],c3);plot([0 1 1 0 0],[0 0 1 1 0]);disp('Weights');
  "IW{1,1}(91,:)'" : Constant  Value=[0.1842627185309813342417584181021084077656269073486328125;-2.128176797157922184311473756679333746433258056640625;-0.2361964893001895493540587267489172518253326416015625;1.3462800682363627036153275184915401041507720947265625;-0.391289828652010285292561775349895469844341278076171875;1.8321318413749632103559861207031644880771636962890625;-5.91451439891542651849931644392199814319610595703125;-1.71524544678979840028887338121421635150909423828125;4.50818118422850222515307905268855392932891845703125]
      mask Display: e = 0.06;c1 = [120 150 230]/255;c2 = ([120 150 230]+0)/383;c3 = ([120 150 230]+128)/383;patch([0 1 1 0],[0 0 1 1],c1);patch([0 1 1 1-e 1-e 0+e],[0 0 1 1-e 0+e 0+e],c2);patch([0 0 1 1-e 0+e 0+e],[0 1 1 1-e 1-e 0+e],c3);plot([0 1 1 0 0],[0 0 1 1 0]);disp('Weights');
  "IW{1,1}(92,:)'" : Constant  Value=[0.3552982777562323501996388586121611297130584716796875;0.4630661803337894344423375514452345669269561767578125;1.2942875819770229828264973548357374966144561767578125;-0.1633050610546715464277411911098170094192028045654296875;0.7230808954060579107903095064102672040462493896484375;-1.2965439882980243080368154551251791417598724365234375;3.2245056324802643388238720945082604885101318359375;0.64487842270952511203319090782315470278263092041015625;1.5851869719329496621895714270067401230335235595703125]
      mask Display: e = 0.06;c1 = [120 150 230]/255;c2 = ([120 150 230]+0)/383;c3 = ([120 150 230]+128)/383;patch([0 1 1 0],[0 0 1 1],c1);patch([0 1 1 1-e 1-e 0+e],[0 0 1 1-e 0+e 0+e],c2);patch([0 0 1 1-e 0+e 0+e],[0 1 1 1-e 1-e 0+e],c3);plot([0 1 1 0 0],[0 0 1 1 0]);disp('Weights');
  "IW{1,1}(93,:)'" : Constant  Value=[-2.225224899470779948984500151709653437137603759765625;-2.03931748028635961844656776520423591136932373046875;-0.47317520842780869116950270836241543292999267578125;3.147668454354726197408353982609696686267852783203125;3.37075324673446541368093676283024251461029052734375;2.708250821553130460728198158903978765010833740234375;6.23915883008200555792654995457269251346588134765625;2.3278023042991566882164988783188164234161376953125;3.45233573415150640784077040734700858592987060546875]
      mask Display: e = 0.06;c1 = [120 150 230]/255;c2 = ([120 150 230]+0)/383;c3 = ([120 150 230]+128)/383;patch([0 1 1 0],[0 0 1 1],c1);patch([0 1 1 1-e 1-e 0+e],[0 0 1 1-e 0+e 0+e],c2);patch([0 0 1 1-e 0+e 0+e],[0 1 1 1-e 1-e 0+e],c3);plot([0 1 1 0 0],[0 0 1 1 0]);disp('Weights');
  "IW{1,1}(94,:)'" : Constant  Value=[-0.8093553134919961866700077735004015266895294189453125;0.77982683431906618665152564062736928462982177734375;0.82063649586372078292839660207391716539859771728515625;0.61936253163637855490009087588987313210964202880859375;0.9405029540089604456198912885156460106372833251953125;1.4069653562309827332654776910203509032726287841796875;0.64897693350145047030963496581534855067729949951171875;-0.313206641156959786354008201669785194098949432373046875;-0.1744209234017403409300328576136962510645389556884765625]
      mask Display: e = 0.06;c1 = [120 150 230]/255;c2 = ([120 150 230]+0)/383;c3 = ([120 150 230]+128)/383;patch([0 1 1 0],[0 0 1 1],c1);patch([0 1 1 1-e 1-e 0+e],[0 0 1 1-e 0+e 0+e],c2);patch([0 0 1 1-e 0+e 0+e],[0 1 1 1-e 1-e 0+e],c3);plot([0 1 1 0 0],[0 0 1 1 0]);disp('Weights');
  "IW{1,1}(95,:)'" : Constant  Value=[1.453130416013045600465147799695841968059539794921875;2.33287198139894069726096859085373580455780029296875;0.59688948284861975679405077244155108928680419921875;-0.4386983185674486751537415329948998987674713134765625;1.5617555063256685077277552409213967621326446533203125;0.250200502195142282513273812583065591752529144287109375;1.6372966711740122303098132761078886687755584716796875;0.94919275940891589815606721458607353270053863525390625;0.2049894899036105722078815460918121971189975738525390625]
      mask Display: e = 0.06;c1 = [120 150 230]/255;c2 = ([120 150 230]+0)/383;c3 = ([120 150 230]+128)/383;patch([0 1 1 0],[0 0 1 1],c1);patch([0 1 1 1-e 1-e 0+e],[0 0 1 1-e 0+e 0+e],c2);patch([0 0 1 1-e 0+e 0+e],[0 1 1 1-e 1-e 0+e],c3);plot([0 1 1 0 0],[0 0 1 1 0]);disp('Weights');
  "IW{1,1}(96,:)'" : Constant  Value=[0.0930250898478679477676678288844414055347442626953125;-1.54351827077867387316700842347927391529083251953125;-1.0069685014582281379347250549471937119960784912109375;-0.07113178434126658788994035376163083128631114959716796875;-0.3612640308372052633245630204328335821628570556640625;0.2936818288635334450731306787929497659206390380859375;-0.05569788749437724895141599290582234971225261688232421875;0.305064227242055618916083403746597468852996826171875;-2.20276663220090451744681558921001851558685302734375]
      mask Display: e = 0.06;c1 = [120 150 230]/255;c2 = ([120 150 230]+0)/383;c3 = ([120 150 230]+128)/383;patch([0 1 1 0],[0 0 1 1],c1);patch([0 1 1 1-e 1-e 0+e],[0 0 1 1-e 0+e 0+e],c2);patch([0 0 1 1-e 0+e 0+e],[0 1 1 1-e 1-e 0+e],c3);plot([0 1 1 0 0],[0 0 1 1 0]);disp('Weights');
  "IW{1,1}(97,:)'" : Constant  Value=[1.37164238005714356205544390832073986530303955078125;-0.07933477577610571762622981850654468871653079986572265625;-0.459087043910794634360428290165145881474018096923828125;1.7075685327056528972633486773702315986156463623046875;0.7830262410438704190340786226443015038967132568359375;-0.5167610370100259586934043909423053264617919921875;-0.780016292146436196475178803666494786739349365234375;2.21441091096581121888675625086762011051177978515625;-2.04757683102025733745676916441880166530609130859375]
      mask Display: e = 0.06;c1 = [120 150 230]/255;c2 = ([120 150 230]+0)/383;c3 = ([120 150 230]+128)/383;patch([0 1 1 0],[0 0 1 1],c1);patch([0 1 1 1-e 1-e 0+e],[0 0 1 1-e 0+e 0+e],c2);patch([0 0 1 1-e 0+e 0+e],[0 1 1 1-e 1-e 0+e],c3);plot([0 1 1 0 0],[0 0 1 1 0]);disp('Weights');
  "IW{1,1}(98,:)'" : Constant  Value=[-7.1412377312193502376658216235227882862091064453125;-7.4202126710954257049479565466754138469696044921875;-8.80393114661506359652776154689490795135498046875;-6.703727992005685365484168869443237781524658203125;-8.2337452620168125605459863436408340930938720703125;-7.25055868318500262859060967457480728626251220703125;-8.4275544081344602176386615610681474208831787109375;-7.765276442462489825402371934615075588226318359375;-8.823558118163031593894629622809588909149169921875]
      mask Display: e = 0.06;c1 = [120 150 230]/255;c2 = ([120 150 230]+0)/383;c3 = ([120 150 230]+128)/383;patch([0 1 1 0],[0 0 1 1],c1);patch([0 1 1 1-e 1-e 0+e],[0 0 1 1-e 0+e 0+e],c2);patch([0 0 1 1-e 0+e 0+e],[0 1 1 1-e 1-e 0+e],c3);plot([0 1 1 0 0],[0 0 1 1 0]);disp('Weights');
  "IW{1,1}(99,:)'" : Constant  Value=[0.11834596110366658872070644292762153781950473785400390625;0.427360129427146351321908923637238331139087677001953125;0.74260668796197937258085630674031563103199005126953125;-0.64611809440997813869245192108792252838611602783203125;-1.374667449125010154631354453158564865589141845703125;-1.2546649455115381766034943211707286536693572998046875;-0.004488999004754942560857511324456936563365161418914794921875;-0.87626664295376688329497483209706842899322509765625;-0.16874075802749277652736736854421906173229217529296875]
      mask Display: e = 0.06;c1 = [120 150 230]/255;c2 = ([120 150 230]+0)/383;c3 = ([120 150 230]+128)/383;patch([0 1 1 0],[0 0 1 1],c1);patch([0 1 1 1-e 1-e 0+e],[0 0 1 1-e 0+e 0+e],c2);patch([0 0 1 1-e 0+e 0+e],[0 1 1 1-e 1-e 0+e],c3);plot([0 1 1 0 0],[0 0 1 1 0]);disp('Weights');
  Mux : Mux  Inputs=100
      mask Display: e = 0.06;c1 = [120 150 230]/255;c2 = ([120 150 230]+0)/383;c3 = ([120 150 230]+128)/383;patch([0 1 1 0],[0 0 1 1],c1);patch([0 1 1 1-e 1-e 0+e],[0 0 1 1-e 0+e 0+e],c2);patch([0 0 1 1-e 0+e 0+e],[0 1 1 1-e 1-e 0+e],c3);plot([0 1 1 0 0],[0 0 1 1 0]);disp('Mux');
  dotprod{1..100} (100 alike) : neural/Weight Functions/dotprod
  "iz{1,1}" : Outport
      mask Display: e = 0.06;c1 = [120 230 180]/255;c2 = ([120 230 180]+0)/(256+128);c3 = ([120 230 180]+128)/(256+128);patch([0 1 1 0],[0 0 1 1],c1);patch([0 1 1 1-e 1-e 0+e],[0 0 1 1-e 0+e 0+e],c2);patch([0 0 1 1-e 0+e 0+e],[0 1 1 1-e 1-e 0+e],c3);plot([0 1 1 0 0],[0 0 1 1 0]);
  wires:
  "IW{1,1}(1,:)'"/1 -> dotprod1/1
  "pd{1,1}"/1 -> dotprod1/2, dotprod2/2, dotprod3/2, dotprod4/2, dotprod5/2, dotprod6/2, dotprod7/2, dotprod8/2, dotprod9/2, dotprod10/2, dotprod11/2, dotprod12/2, dotprod13/2, dotprod14/2, dotprod15/2, dotprod16/2, dotprod17/2, dotprod18/2, dotprod19/2, dotprod20/2, dotprod21/2, dotprod22/2, dotprod23/2, dotprod24/2, dotprod25/2, dotprod26/2, dotprod27/2, dotprod28/2, dotprod29/2, dotprod30/2, dotprod31/2, dotprod32/2, dotprod33/2, dotprod34/2, dotprod35/2, dotprod36/2, dotprod37/2, dotprod38/2, dotprod39/2, dotprod40/2, dotprod41/2, dotprod42/2, dotprod43/2, dotprod44/2, dotprod45/2, dotprod46/2, dotprod47/2, dotprod48/2, dotprod49/2, dotprod50/2, dotprod51/2, dotprod52/2, dotprod53/2, dotprod54/2, dotprod55/2, dotprod56/2, dotprod57/2, dotprod58/2, dotprod59/2, dotprod60/2, dotprod61/2, dotprod62/2, dotprod63/2, dotprod64/2, dotprod65/2, dotprod66/2, dotprod67/2, dotprod68/2, dotprod69/2, dotprod70/2, dotprod71/2, dotprod72/2, dotprod73/2, dotprod74/2, dotprod75/2, dotprod76/2, dotprod77/2, dotprod78/2, dotprod79/2, dotprod80/2, dotprod81/2, dotprod82/2, dotprod83/2, dotprod84/2, dotprod85/2, dotprod86/2, dotprod87/2, dotprod88/2, dotprod89/2, dotprod90/2, dotprod91/2, dotprod92/2, dotprod93/2, dotprod94/2, dotprod95/2, dotprod96/2, dotprod97/2, dotprod98/2, dotprod99/2, dotprod100/2
  dotprod1/1 -> Mux/1
  "IW{1,1}(2,:)'"/1 -> dotprod2/1
  dotprod2/1 -> Mux/2
  "IW{1,1}(3,:)'"/1 -> dotprod3/1
  dotprod3/1 -> Mux/3
  "IW{1,1}(4,:)'"/1 -> dotprod4/1
  dotprod4/1 -> Mux/4
  "IW{1,1}(5,:)'"/1 -> dotprod5/1
  dotprod5/1 -> Mux/5
  "IW{1,1}(6,:)'"/1 -> dotprod6/1
  dotprod6/1 -> Mux/6
  "IW{1,1}(7,:)'"/1 -> dotprod7/1
  dotprod7/1 -> Mux/7
  "IW{1,1}(8,:)'"/1 -> dotprod8/1
  dotprod8/1 -> Mux/8
  "IW{1,1}(9,:)'"/1 -> dotprod9/1
  dotprod9/1 -> Mux/9
  "IW{1,1}(10,:)'"/1 -> dotprod10/1
  dotprod10/1 -> Mux/10
  "IW{1,1}(11,:)'"/1 -> dotprod11/1
  dotprod11/1 -> Mux/11
  "IW{1,1}(12,:)'"/1 -> dotprod12/1
  dotprod12/1 -> Mux/12
  "IW{1,1}(13,:)'"/1 -> dotprod13/1
  dotprod13/1 -> Mux/13
  "IW{1,1}(14,:)'"/1 -> dotprod14/1
  dotprod14/1 -> Mux/14
  "IW{1,1}(15,:)'"/1 -> dotprod15/1
  dotprod15/1 -> Mux/15
  "IW{1,1}(16,:)'"/1 -> dotprod16/1
  dotprod16/1 -> Mux/16
  "IW{1,1}(17,:)'"/1 -> dotprod17/1
  dotprod17/1 -> Mux/17
  "IW{1,1}(18,:)'"/1 -> dotprod18/1
  dotprod18/1 -> Mux/18
  "IW{1,1}(19,:)'"/1 -> dotprod19/1
  dotprod19/1 -> Mux/19
  "IW{1,1}(20,:)'"/1 -> dotprod20/1
  dotprod20/1 -> Mux/20
  "IW{1,1}(21,:)'"/1 -> dotprod21/1
  dotprod21/1 -> Mux/21
  "IW{1,1}(22,:)'"/1 -> dotprod22/1
  dotprod22/1 -> Mux/22
  "IW{1,1}(23,:)'"/1 -> dotprod23/1
  dotprod23/1 -> Mux/23
  "IW{1,1}(24,:)'"/1 -> dotprod24/1
  dotprod24/1 -> Mux/24
  "IW{1,1}(25,:)'"/1 -> dotprod25/1
  dotprod25/1 -> Mux/25
  "IW{1,1}(26,:)'"/1 -> dotprod26/1
  dotprod26/1 -> Mux/26
  "IW{1,1}(27,:)'"/1 -> dotprod27/1
  dotprod27/1 -> Mux/27
  "IW{1,1}(28,:)'"/1 -> dotprod28/1
  dotprod28/1 -> Mux/28
  "IW{1,1}(29,:)'"/1 -> dotprod29/1
  dotprod29/1 -> Mux/29
  "IW{1,1}(30,:)'"/1 -> dotprod30/1
  dotprod30/1 -> Mux/30
  "IW{1,1}(31,:)'"/1 -> dotprod31/1
  dotprod31/1 -> Mux/31
  "IW{1,1}(32,:)'"/1 -> dotprod32/1
  dotprod32/1 -> Mux/32
  "IW{1,1}(33,:)'"/1 -> dotprod33/1
  dotprod33/1 -> Mux/33
  "IW{1,1}(34,:)'"/1 -> dotprod34/1
  dotprod34/1 -> Mux/34
  "IW{1,1}(35,:)'"/1 -> dotprod35/1
  dotprod35/1 -> Mux/35
  "IW{1,1}(36,:)'"/1 -> dotprod36/1
  dotprod36/1 -> Mux/36
  "IW{1,1}(37,:)'"/1 -> dotprod37/1
  dotprod37/1 -> Mux/37
  "IW{1,1}(38,:)'"/1 -> dotprod38/1
  dotprod38/1 -> Mux/38
  "IW{1,1}(39,:)'"/1 -> dotprod39/1
  dotprod39/1 -> Mux/39
  "IW{1,1}(40,:)'"/1 -> dotprod40/1
  dotprod40/1 -> Mux/40
  "IW{1,1}(41,:)'"/1 -> dotprod41/1
  dotprod41/1 -> Mux/41
  "IW{1,1}(42,:)'"/1 -> dotprod42/1
  dotprod42/1 -> Mux/42
  "IW{1,1}(43,:)'"/1 -> dotprod43/1
  dotprod43/1 -> Mux/43
  "IW{1,1}(44,:)'"/1 -> dotprod44/1
  dotprod44/1 -> Mux/44
  "IW{1,1}(45,:)'"/1 -> dotprod45/1
  dotprod45/1 -> Mux/45
  "IW{1,1}(46,:)'"/1 -> dotprod46/1
  dotprod46/1 -> Mux/46
  "IW{1,1}(47,:)'"/1 -> dotprod47/1
  dotprod47/1 -> Mux/47
  "IW{1,1}(48,:)'"/1 -> dotprod48/1
  dotprod48/1 -> Mux/48
  "IW{1,1}(49,:)'"/1 -> dotprod49/1
  dotprod49/1 -> Mux/49
  "IW{1,1}(50,:)'"/1 -> dotprod50/1
  dotprod50/1 -> Mux/50
  "IW{1,1}(51,:)'"/1 -> dotprod51/1
  dotprod51/1 -> Mux/51
  "IW{1,1}(52,:)'"/1 -> dotprod52/1
  dotprod52/1 -> Mux/52
  "IW{1,1}(53,:)'"/1 -> dotprod53/1
  dotprod53/1 -> Mux/53
  "IW{1,1}(54,:)'"/1 -> dotprod54/1
  dotprod54/1 -> Mux/54
  "IW{1,1}(55,:)'"/1 -> dotprod55/1
  dotprod55/1 -> Mux/55
  "IW{1,1}(56,:)'"/1 -> dotprod56/1
  dotprod56/1 -> Mux/56
  "IW{1,1}(57,:)'"/1 -> dotprod57/1
  dotprod57/1 -> Mux/57
  "IW{1,1}(58,:)'"/1 -> dotprod58/1
  dotprod58/1 -> Mux/58
  "IW{1,1}(59,:)'"/1 -> dotprod59/1
  dotprod59/1 -> Mux/59
  "IW{1,1}(60,:)'"/1 -> dotprod60/1
  dotprod60/1 -> Mux/60
  "IW{1,1}(61,:)'"/1 -> dotprod61/1
  dotprod61/1 -> Mux/61
  "IW{1,1}(62,:)'"/1 -> dotprod62/1
  dotprod62/1 -> Mux/62
  "IW{1,1}(63,:)'"/1 -> dotprod63/1
  dotprod63/1 -> Mux/63
  "IW{1,1}(64,:)'"/1 -> dotprod64/1
  dotprod64/1 -> Mux/64
  "IW{1,1}(65,:)'"/1 -> dotprod65/1
  dotprod65/1 -> Mux/65
  "IW{1,1}(66,:)'"/1 -> dotprod66/1
  dotprod66/1 -> Mux/66
  "IW{1,1}(67,:)'"/1 -> dotprod67/1
  dotprod67/1 -> Mux/67
  "IW{1,1}(68,:)'"/1 -> dotprod68/1
  dotprod68/1 -> Mux/68
  "IW{1,1}(69,:)'"/1 -> dotprod69/1
  dotprod69/1 -> Mux/69
  "IW{1,1}(70,:)'"/1 -> dotprod70/1
  dotprod70/1 -> Mux/70
  "IW{1,1}(71,:)'"/1 -> dotprod71/1
  dotprod71/1 -> Mux/71
  "IW{1,1}(72,:)'"/1 -> dotprod72/1
  dotprod72/1 -> Mux/72
  "IW{1,1}(73,:)'"/1 -> dotprod73/1
  dotprod73/1 -> Mux/73
  "IW{1,1}(74,:)'"/1 -> dotprod74/1
  dotprod74/1 -> Mux/74
  "IW{1,1}(75,:)'"/1 -> dotprod75/1
  dotprod75/1 -> Mux/75
  "IW{1,1}(76,:)'"/1 -> dotprod76/1
  dotprod76/1 -> Mux/76
  "IW{1,1}(77,:)'"/1 -> dotprod77/1
  dotprod77/1 -> Mux/77
  "IW{1,1}(78,:)'"/1 -> dotprod78/1
  dotprod78/1 -> Mux/78
  "IW{1,1}(79,:)'"/1 -> dotprod79/1
  dotprod79/1 -> Mux/79
  "IW{1,1}(80,:)'"/1 -> dotprod80/1
  dotprod80/1 -> Mux/80
  "IW{1,1}(81,:)'"/1 -> dotprod81/1
  dotprod81/1 -> Mux/81
  "IW{1,1}(82,:)'"/1 -> dotprod82/1
  dotprod82/1 -> Mux/82
  "IW{1,1}(83,:)'"/1 -> dotprod83/1
  dotprod83/1 -> Mux/83
  "IW{1,1}(84,:)'"/1 -> dotprod84/1
  dotprod84/1 -> Mux/84
  "IW{1,1}(85,:)'"/1 -> dotprod85/1
  dotprod85/1 -> Mux/85
  "IW{1,1}(86,:)'"/1 -> dotprod86/1
  dotprod86/1 -> Mux/86
  "IW{1,1}(87,:)'"/1 -> dotprod87/1
  dotprod87/1 -> Mux/87
  "IW{1,1}(88,:)'"/1 -> dotprod88/1
  dotprod88/1 -> Mux/88
  "IW{1,1}(89,:)'"/1 -> dotprod89/1
  dotprod89/1 -> Mux/89
  "IW{1,1}(90,:)'"/1 -> dotprod90/1
  dotprod90/1 -> Mux/90
  "IW{1,1}(91,:)'"/1 -> dotprod91/1
  dotprod91/1 -> Mux/91
  "IW{1,1}(92,:)'"/1 -> dotprod92/1
  dotprod92/1 -> Mux/92
  "IW{1,1}(93,:)'"/1 -> dotprod93/1
  dotprod93/1 -> Mux/93
  "IW{1,1}(94,:)'"/1 -> dotprod94/1
  dotprod94/1 -> Mux/94
  "IW{1,1}(95,:)'"/1 -> dotprod95/1
  dotprod95/1 -> Mux/95
  "IW{1,1}(96,:)'"/1 -> dotprod96/1
  dotprod96/1 -> Mux/96
  "IW{1,1}(97,:)'"/1 -> dotprod97/1
  dotprod97/1 -> Mux/97
  "IW{1,1}(98,:)'"/1 -> dotprod98/1
  dotprod98/1 -> Mux/98
  "IW{1,1}(99,:)'"/1 -> dotprod99/1
  dotprod99/1 -> Mux/99
  "IW{1,1}(100,:)'"/1 -> dotprod100/1
  dotprod100/1 -> Mux/100
  Mux/1 -> "iz{1,1}"/1
